simulink model "acf_rl_native"  (R2026b)
settings: Solver=ode4  StopTime=inf  FixedStep=3.3333333333333333e-06
InitFcn:
  | acf_select_actuator(bdroot);
model workspace (MAT data in the model file):
  acfControlVersion = 'force-observer-v1'
  acfImplementation = 'simple'
  acfLayoutVersion = 1
  p : object (value not decoded)
  pCompliant.actuator.kind = 'voice_coil'
  pCompliant.sim.step = 5e-05
  pCompliant.sim.stopTime = 4
  pCompliant.sim.evaluateFrom = 0
  pCompliant.force.reference = 20
  pCompliant.force.tolerance = 0.5
  pCompliant.force.sampleTime = 0.0001
  pCompliant.force.antiWindupRate = 30
  pCompliant.force.derivativeFilter = 0.001
  pCompliant.mechanics.mA = 0.4
  pCompliant.mechanics.mB = 0.6
  pCompliant.mechanics.mS = 1.4
  pCompliant.mechanics.k1 = 19746
  pCompliant.mechanics.k2 = 19746
  pCompliant.mechanics.c1 = 30
  pCompliant.mechanics.c2 = 5
  pCompliant.mechanics.gravity = 9.81
  pCompliant.mechanics.angle = 0
  pCompliant.mechanics.travelMin = 0
  pCompliant.mechanics.travelMax = 0.025
  pCompliant.mechanics.midTravel = 0.0125
  pCompliant.mechanics.lowerRigid = 0
  pCompliant.mechanics.upperRigid = 0
  pCompliant.robot.initialExcessForce = 10
  pCompliant.robot.sampleTime = 0.01
  pCompliant.robot.delay = 0.08
  pCompliant.robot.recenterGain = 0.8
  pCompliant.robot.deadband = 0.0005
  pCompliant.robot.responseTime = 0.06
  pCompliant.robot.maxSpeed = 0.02
  pCompliant.robot.maxAcceleration = 0.5
  pCompliant.robot.nominalVelocity = 0.005
  pCompliant.robot.errorRiseTime = 0.2
  pCompliant.robot.errorForce = 20
  pCompliant.robot.forceGate.enabled = 1
  pCompliant.robot.forceGate.errorBand_N = 0.2
  pCompliant.robot.forceGate.maxRate_N_s = 2
  pCompliant.robot.forceGate.dwellTime = 0.1
  pCompliant.robot.forceGate.filterTime = 0.1
  pCompliant.robot.forceGate.maxDelayGainProduct = 0.25
  pCompliant.robot.initialPositionOffset_m = 0
  pCompliant.sensor.sampleTime = 0.0001
  pCompliant.sensor.filterTime = 0.0001
  pCompliant.sensor.delay = 0.0001
  pCompliant.sensor.bias = 0
  pCompliant.sensor.noiseRms = 0.02
  pCompliant.sensor.seed = 1729
  pCompliant.sensor.strokeNoiseRms = 1e-06
  pCompliant.sensor.strokeDelay = 0.0001
  pCompliant.sensor.distalMass_kg = 1.4
  pCompliant.sensor.distalMass_model_kg = 1.4
  pCompliant.sensor.strokeBias = 0
  pCompliant.sensor.positionTarget = 'tool_relative_A'
  pCompliant.sensor.positionModel = 1
  pCompliant.surface.kind = 'sharp_bump'
  pCompliant.surface.startTime = 2
  pCompliant.surface.height = 0.001
  pCompliant.surface.width = 0.01
  pCompliant.surface.scanSpeed = 0.1
  pCompliant.surface.repeatPeriod = 1.2
  pCompliant.screw.lead = 0.01
  pCompliant.screw.rotorInertia = 5e-06
  pCompliant.screw.torqueConstant = 0.05
  pCompliant.screw.backEmfConstant = 0.05
  pCompliant.screw.resistance = 1
  pCompliant.screw.inductance = 0.001
  pCompliant.screw.peakCurrent = 5
  pCompliant.screw.voltage = 36
  pCompliant.screw.currentResponse = 0.001
  pCompliant.screw.coulombTorque = 0.004
  pCompliant.screw.viscousTorque = 2e-05
  pCompliant.screw.frictionSpeed = 0.2
  pCompliant.screw.speedBandwidth = 600
  pCompliant.screw.speedDamping = 1
  pCompliant.screw.speedAntiWindup = 100
  pCompliant.screw.maxLinearSpeedRequest = 0.1
  pCompliant.screw.forceKp = 0.08
  pCompliant.screw.forceKi = 0.5
  pCompliant.screw.forceKd = 0
  pCompliant.coil.forceConstant = 20
  pCompliant.coil.resistance = 4
  pCompliant.coil.inductance = 0.003
  pCompliant.coil.peakCurrent = 3.5
  pCompliant.coil.voltage = 24
  pCompliant.coil.currentResponse = 0.0001
  pCompliant.coil.coulombForce = 0.2
  pCompliant.coil.viscousFriction = 2
  pCompliant.coil.frictionSpeed = 0.0002
  pCompliant.coil.control.forceScale_N = 0.08
  pCompliant.coil.control.integralScale_Ns = 0.02
  pCompliant.coil.control.velocityScale_m_s = 0.1
  pCompliant.coil.control.currentScale_A = 1
  pCompliant.coil.control.surfaceJerkPower = 30
  pCompliant.coil.control.robotJerkPower = 0.2
  pCompliant.coil.control.forceNoise_N = 0.06
  pCompliant.coil.control.strokeNoise_m = 1e-06
  pCompliant.coil.control.frictionPower = 0.0009
  pCompliant.coil.strategy = 'observer'
  pCompliant.coil.forceKp = 0.03
  pCompliant.coil.forceKi = 20
  pCompliant.coil.forceKd = 5e-06
  pCompliant.coil.derivativeFilter = 0.0003
  pCompliant.coil.directCoulombCorrection = 1
  pCompliant.ideal.positionGain = 100
  pCompliant.ideal.velocityTime = 0.005
  pCompliant.ideal.maxSpeed = 0.1
  pCompliant.ideal.maxAcceleration = 20
  pCompliant.ideal.maxAxialForce = Inf
  pCompliant.ideal.forceKp = 7.49999999996e-05
  pCompliant.ideal.forceKi = 0.0179999999999
  pCompliant.ideal.forceKd = 0
  pCompliant.d.M = 1
  pCompliant.d.alpha = 0.4
  pCompliant.d.beta = 0.6
  pCompliant.d.mu = 0.24
  pCompliant.d.g = 9.81
  pCompliant.d.keq = 9873
  pCompliant.d.ell = 0.00159154943092
  pCompliant.d.q10 = 6.266
  pCompliant.d.q20 = -3.544
  pCompliant.d.holdForce = 0.38
  pCompliant.d.r0 = -0.00101286336473
  pCompliant.d.u0 = -0.00101286336473
  pCompliant.d.z0 = -0.000405145345893
  pCompliant.d.forceTicks = 2
  pCompliant.d.sensorTicks = 2
  pCompliant.d.robotTicks = 200
  pCompliant.d.sensorDelaySamples = 1
  pCompliant.d.robotDelaySamples = 8
  pCompliant.d.strokeDelaySamples = 1
  pCompliant.d.duration = 0.1
  pCompliant.d.screwHoldCurrent = 0.012095775675
  pCompliant.d.coilHoldCurrent = 0.019
  pCompliant.d.speedKp = 0.134590250444
  pCompliant.d.speedKi = 40.3770751333
  pCompliant.d.forceKp = 0.03
  pCompliant.d.forceKi = 20
  pCompliant.d.forceFeedforward = 0.019
  pCompliant.d.commandMax = 3.5
  pCompliant.d.commandMin = -3.5
  pCompliant.d.coilControl.A = [0.999835746645  0.00997449730862  2.7375365216e-08  7.61651197841e-10  0  -1.6633847877e-06  0.000122366168772  4.99154092539e-05  -1.86997975018e-12  -0.00413675380364  0.0458269373325; -0.0328205964433  0.994849329683  8.20753911342e-06  2.35203256889e-07  0  -0.000332344666304  0.0209978497532  0.00997449730862  -7.61339530061e-10  -0.0648188925165  1.4845666459; 2.73753650079e-08  4.2275891689e-09  0.999753329061  0.00999293153119  0  -2.49816229398e-06  0.000183793671919  1.05385993767e-11  -4.99493633224e-05  -0.00412753174604  0.239523975118; 8.20753911342e-06  1.27434271721e-06  -0.0493177743256  0.99850452489  0  -0.000499438537288  0.0315644865369  4.22758920489e-09  -0.00998460663731  -0.0815985605483  3.59792231768; -0.00016422598009  -2.54984637932e-05  -0.000246643563285  -7.06770715559e-06  1  0.00999583845292  0.000306159840692  -8.45802075454e-08  2.28686000246e-08  -0.00684940440528  0.403167864802; -0.0328123889042  -0.00514939597465  -0.0493095667865  -0.00149523990651  0  0.999168216796  0.05256233629  -2.54984637932e-05  7.06389572225e-06  -0.13409460151  6.02904033295; 0  0  0  0  0  0  0.367879441171  0  0  -7.97431898094e-16  1.21101563191e-14; 0  0  0  0  0  0  0  1  0  -0.0527908571517  -3.83687930661; 0  0  0  0  0  0  0  0  0.998334721451  -1.1298863089e-06  6.97113672767e-05; 12.4818525546  1.89636167649  0  0  0  0  0  0  0  0.118421048821  5.02664399852; 1  0  0  0  -1  0  0  0  0  0.00201545569863  -0.311994254342]
  pCompliant.d.coilControl.B = [0.00413675380364  -45.8269373325  4.39723099978e-05  -8.31692393848e-06  -1.87066620522e-13; 0.0648188925165  -1484.5666459  0.0122366168773  -0.00166172333152  -7.61651187423e-11; 0.00412753174604  -239.523975118  6.60225574786e-05  -1.24908114699e-05  -4.99771201703e-06; 0.0815985605483  -3597.92231768  0.018379367192  -0.00249719268644  -0.000999293153119; 0.00684940440528  -403.167864802  0.000109994867477  -2.08077354085e-05  2.28779591191e-09; 0.13409460151  -6029.04033295  0.0306159840692  -0.00415891601796  7.06770715559e-07; 7.97431898094e-16  -1.21101563191e-11  0.632120558829  0  0; 0.0527908571517  3836.87930661  0  0  0; 1.1298863089e-06  -0.0697113672767  0  0  0; 0.24945839235  -5026.64399852  0  0  0; -0.00201545569863  311.994254342  0  0  0]
  pCompliant.d.coilControl.C = [0.001  0  0  0  0  0  0  0  0  -3.48871506098e-06  3.07351175913e-05; 0  0.1  0  0  0  0  0  0  0  -0.00647853206073  0.153375714294; 0  0  0.001  0  0  0  0  0  0  -3.3097478138e-06  0.000203450968232; 0  0  0  0.1  0  0  0  0  0  -0.00819516417082  0.361638855458; 0  0  0  0  0.001  0  0  0  0  -5.5041707596e-06  0.000342729371933; 0  0  0  0  0  0.1  0  0  0  -0.0134942008024  0.605832757613; 0  0  0  0  0  0  1  0  0  -2.16764463802e-15  3.2918817862e-14; 0  0  0  0  0  0  0  10  0  -0.527908571517  -38.3687930661; 0  0  0  0  0  0  0  0  10  -1.13177102291e-05  0.00069827649764]
  pCompliant.d.coilControl.D = [3.48871506098e-06  -0.0307351175913  0  0  0; 0.00647853206073  -153.375714294  0  0  0; 3.3097478138e-06  -0.203450968232  0  0  0; 0.00819516417082  -361.638855458  0  0  0; 5.5041707596e-06  -0.342729371933  0  0  0; 0.0134942008024  -605.832757613  0  0  0; 2.16764463802e-15  -3.2918817862e-11  0  0  0; 0.527908571517  38368.7930661  0  0  0; 1.13177102291e-05  -0.69827649764  0  0  0]
  pCompliant.d.coilControl.feedback = [-244976.099879 -409.158583232 -93.7245887968 0.421195616079 0 0 -0.929640363397 -17.5713692327 -0.00189860404734]
  pCompliant.d.coilControl.integralGain = 50
  pCompliant.d.coilControl.force = [19746 30 0 0 0 0 0 1.4 0]
  pCompliant.d.recenterGain = 0.735294117647
  pCompliant.d.positionMeasurementBias = -0.0135128633647
  pCompliant.d.positionMeasurementInitial = 0.0135128633647
  pCompliant.d.forceKd = 0
  pCompliant.d.derivativeFilter = 0.0003
  pCompliant.springs.maxCombinedLength_m = 0.1
  pCompliant.springs.commonPreload_N = 34
  pCompliant.springs.workingClearance_m = 0.0005
  pCompliant.springs.unseatingClearance_m = 0.00025
  pCompliant.springs.lower.part = 'D-180S'
  pCompliant.springs.lower.rate_N_m = 9873
  pCompliant.springs.lower.freeLength_m = 0.0181
  pCompliant.springs.lower.freeLengthTolerance_m = 0.00049
  pCompliant.springs.lower.minWorkingLength_m = 0.01055
  pCompliant.springs.lower.maxCyclicStroke_m = 0.00318
  pCompliant.springs.lower.forceEnvelope_N = 68.543
  pCompliant.springs.upper.part = 'D-180S'
  pCompliant.springs.upper.rate_N_m = 9873
  pCompliant.springs.upper.freeLength_m = 0.0181
  pCompliant.springs.upper.freeLengthTolerance_m = 0.00049
  pCompliant.springs.upper.minWorkingLength_m = 0.01055
  pCompliant.springs.upper.maxCyclicStroke_m = 0.00318
  pCompliant.springs.upper.forceEnvelope_N = 68.543
  pCompliant.robotPrediction.enabled = 1
  pCompliant.robotPrediction.delay = 0.08
  pCompliant.robotPrediction.responseTime = 0.06
  pCompliant.robotPrediction.maxSpeed = 0.02
  pCompliant.robotPrediction.maxAcceleration = 0.5
  pCompliant.robotPrediction.residualTime = 0.06
  pCompliant.robotPrediction.residualJerkPower = 0.0002
  pCompliant.robotPrediction.boundedNominalPath = 1
  pCompliant.robotPrediction.delaySamples = 8
  pCompliant.robotPrediction.surfaceJerkEnabled = 0
  pCompliant.robotPrediction.surfaceSnapPower = 1000000
  pCompliant.robotPrediction.surfaceJerkDecayTime = Inf
  pCompliant.robotPrediction.surfaceJerkFeedforwardGain = 0
  pNearContact.actuator.kind = 'voice_coil'
  pNearContact.sim.step = 0.0001
  pNearContact.sim.stopTime = 4
  pNearContact.sim.evaluateFrom = 0
  pNearContact.force.reference = 20
  pNearContact.force.tolerance = 0.5
  pNearContact.force.sampleTime = 0.0002
  pNearContact.force.antiWindupRate = 30
  pNearContact.force.derivativeFilter = 0.001
  pNearContact.mechanics.mA = 0.4
  pNearContact.mechanics.mB = 0.6
  pNearContact.mechanics.mS = 1.4
  pNearContact.mechanics.k1 = 19746
  pNearContact.mechanics.k2 = 0
  pNearContact.mechanics.c1 = 60
  pNearContact.mechanics.c2 = 0
  pNearContact.mechanics.gravity = 9.81
  pNearContact.mechanics.angle = 0
  pNearContact.mechanics.travelMin = 0
  pNearContact.mechanics.travelMax = 0.025
  pNearContact.mechanics.midTravel = 0.0125
  pNearContact.mechanics.lowerRigid = 0
  pNearContact.mechanics.upperRigid = 1
  pNearContact.robot.initialExcessForce = 10
  pNearContact.robot.sampleTime = 0.01
  pNearContact.robot.delay = 0.08
  pNearContact.robot.recenterGain = 0.8
  pNearContact.robot.deadband = 0.0005
  pNearContact.robot.responseTime = 0.06
  pNearContact.robot.maxSpeed = 0.02
  pNearContact.robot.maxAcceleration = 0.5
  pNearContact.robot.nominalVelocity = 0
  pNearContact.robot.errorRiseTime = 0.2
  pNearContact.robot.errorForce = 20
  pNearContact.robot.forceGate.enabled = 1
  pNearContact.robot.forceGate.errorBand_N = 0.2
  pNearContact.robot.forceGate.maxRate_N_s = 2
  pNearContact.robot.forceGate.dwellTime = 0.1
  pNearContact.robot.forceGate.filterTime = 0.02
  pNearContact.robot.forceGate.maxDelayGainProduct = 0.25
  pNearContact.robot.initialPositionOffset_m = 0
  pNearContact.sensor.sampleTime = 0.0002
  pNearContact.sensor.filterTime = 0.0003
  pNearContact.sensor.delay = 0
  pNearContact.sensor.bias = 0
  pNearContact.sensor.noiseRms = 0
  pNearContact.sensor.seed = 1729
  pNearContact.sensor.strokeNoiseRms = 1e-06
  pNearContact.sensor.strokeDelay = 0.0002
  pNearContact.sensor.distalMass_kg = 0
  pNearContact.sensor.distalMass_model_kg = 0
  pNearContact.sensor.positionModel = 0
  pNearContact.sensor.positionTarget = 'magnet_gap'
  pNearContact.surface.kind = 'sharp_bump'
  pNearContact.surface.startTime = 2
  pNearContact.surface.height = 0.001
  pNearContact.surface.width = 0.01
  pNearContact.surface.scanSpeed = 0.1
  pNearContact.surface.repeatPeriod = 1.2
  pNearContact.screw.lead = 0.005
  pNearContact.screw.rotorInertia = 2e-05
  pNearContact.screw.torqueConstant = 0.05
  pNearContact.screw.backEmfConstant = 0.05
  pNearContact.screw.resistance = 1
  pNearContact.screw.inductance = 0.001
  pNearContact.screw.peakCurrent = 3
  pNearContact.screw.voltage = 24
  pNearContact.screw.currentResponse = 0.001
  pNearContact.screw.coulombTorque = 0.004
  pNearContact.screw.viscousTorque = 2e-05
  pNearContact.screw.frictionSpeed = 0.2
  pNearContact.screw.speedBandwidth = 150
  pNearContact.screw.speedDamping = 1
  pNearContact.screw.speedAntiWindup = 100
  pNearContact.screw.maxLinearSpeedRequest = 0.1
  pNearContact.screw.forceKp = 0.02
  pNearContact.screw.forceKi = 0.008
  pNearContact.screw.forceKd = 0
  pNearContact.coil.forceConstant = 20
  pNearContact.coil.resistance = 4
  pNearContact.coil.inductance = 0.003
  pNearContact.coil.peakCurrent = 3
  pNearContact.coil.voltage = 24
  pNearContact.coil.currentResponse = 0.0004
  pNearContact.coil.coulombForce = 0.2
  pNearContact.coil.viscousFriction = 2
  pNearContact.coil.frictionSpeed = 0.0002
  pNearContact.coil.control.forceScale_N = 0.04
  pNearContact.coil.control.integralScale_Ns = 0.02
  pNearContact.coil.control.velocityScale_m_s = 0.1
  pNearContact.coil.control.currentScale_A = 1
  pNearContact.coil.control.surfaceJerkPower = 70
  pNearContact.coil.control.robotJerkPower = 0.2
  pNearContact.coil.control.forceNoise_N = 0.06
  pNearContact.coil.control.strokeNoise_m = 1e-06
  pNearContact.coil.control.frictionPower = 0.0009
  pNearContact.coil.strategy = 'observer'
  pNearContact.coil.forceKp = 0.64
  pNearContact.coil.forceKi = 300
  pNearContact.coil.forceKd = 0.0006
  pNearContact.coil.derivativeFilter = 0.0002
  pNearContact.coil.directCoulombCorrection = 0
  pNearContact.ideal.positionGain = 100
  pNearContact.ideal.velocityTime = 0.005
  pNearContact.ideal.maxSpeed = 0.1
  pNearContact.ideal.maxAcceleration = 20
  pNearContact.ideal.maxAxialForce = Inf
  pNearContact.ideal.forceKp = 7.49999999996e-05
  pNearContact.ideal.forceKi = 0.0179999999999
  pNearContact.ideal.forceKd = 0
  pNearContact.d.M = 1
  pNearContact.d.alpha = 0.4
  pNearContact.d.beta = 0.6
  pNearContact.d.mu = 0.24
  pNearContact.d.g = 9.81
  pNearContact.d.keq = 19746
  pNearContact.d.ell = 0.000795774715459
  pNearContact.d.q10 = 6.266
  pNearContact.d.q20 = -3.544
  pNearContact.d.holdForce = 0.38
  pNearContact.d.r0 = -0.000506431682366
  pNearContact.d.u0 = -0.000506431682366
  pNearContact.d.z0 = -0.000202572672946
  pNearContact.d.forceTicks = 2
  pNearContact.d.sensorTicks = 2
  pNearContact.d.robotTicks = 100
  pNearContact.d.sensorDelaySamples = 0
  pNearContact.d.robotDelaySamples = 8
  pNearContact.d.strokeDelaySamples = 1
  pNearContact.d.duration = 0.1
  pNearContact.d.screwHoldCurrent = 0.00604788783749
  pNearContact.d.coilHoldCurrent = 0.019
  pNearContact.d.speedKp = 0.120911890653
  pNearContact.d.speedKi = 9.06839179896
  pNearContact.d.forceKp = 0.64
  pNearContact.d.forceKi = 300
  pNearContact.d.forceFeedforward = 0.019
  pNearContact.d.commandMax = 3
  pNearContact.d.commandMin = -3
  pNearContact.d.coilControl.A = [1.0026534079  0.0208018967614  0  0  0  -6.62025176034e-06  0.000564047674022  0.00254334714763  -4.42128553796e-08  0.000176714388546  -0.204677748701; -0.237328903655  0.927231856972  0  0  0  -0.00065968023534  0.0518668316835  -0.102292582547  -6.62025176034e-06  -0.00920161779651  -4.36343291704; 0  0  0.818730753078  0  0  0  0  0  0  0  0; 0  0  0  0.818730753078  0  0  0  0  0  0  0; -0.00626191608391  -0.00190710475355  0  0  1  0.0199933797482  0.000564047674022  -0.0039776563872  0.000199955787144  -0.000299685353291  -0.591080531092; -0.205759420553  -0.0631754711644  0  0  0  0.999340319765  0.0518668316835  -0.0999096815332  0.0199933797482  -0.0075146691647  -4.76194052863; -7.21925622066e-14  -2.19363604396e-14  0  0  0  0  0.606530659713  -5.11848410256e-14  0  -3.85768571654e-15  -5.1788789238e-13; -0.870024269621  -0.264364712738  0  0  0  0  0  0.383149003611  0  -0.046490664625  2.07853967939; -0.0101705012363  -0.00309039843096  0  0  0  0  0  -0.00721092967225  1  -0.000543471462297  -0.478477076797; 2.12271455447  0.645005941801  0  0  0  0  0  1.5050138642  0  0.113429491443  -0.281433751395; -0.00276622884074  -0.000840543555375  0  0  1  0  0  -0.00196126829588  0  -0.000147816356165  -0.494907709778]
  pNearContact.d.coilControl.B = [-0.000344192630114  204.677748701  9.79775020114e-05  -3.31012588017e-05  0; 0.017922304215  4363.43291704  0.0141011918506  -0.0032984011767  0; 0  0  0  0  0; 0  0  0  0  0; 0.00058370736421  591.080531092  9.79775020113e-05  -3.31012588017e-05  0; 0.0146365769394  4761.94052863  0.0141011918506  -0.0032984011767  0; 7.5137457898e-15  5.1788789238e-10  0.393469340287  0  0; 0.0905514500813  -2078.53967939  0  0  0; 0.00105853786746  478.477076797  0  0  0; 0.779069518257  281.433751395  0  0  0; 0.000287906948728  494.907709778  0  0  0]
  pNearContact.d.coilControl.C = [0.00100660851405  2.00805653396e-06  0  0  0  0  0  4.6854652459e-06  0  3.53132919675e-07  -0.000115963676268; -0.0157866520328  0.0952030835513  0  0  0  0  0  -0.011192805047  0  -0.000843576404514  -0.450749165677; 0  0  0.001  0  0  0  0  0  0  0  0; 0  0  0  0.1  0  0  0  0  0  0  0; -2.76622884074e-06  -8.40543555375e-07  0  0  0.001  0  0  -1.96126829588e-06  0  -1.47816356165e-07  -0.000494907709778; -0.0143494112594  -0.00436019789102  0  0  0  0.1  0  -0.0101737950791  0  -0.000766775927659  -0.485485893323; -1.19025412896e-13  -3.61669440584e-14  0  0  0  0  1  -8.43895361364e-14  0  -6.36024849654e-15  -8.53852784006e-13; -8.70024269621  -2.64364712738  0  0  0  0  0  3.83149003611  0  -0.46490664625  20.7853967939; -0.101705012363  -0.0309039843096  0  0  0  0  0  -0.0721092967225  10  -0.00543471462297  -4.78477076797]
  pNearContact.d.coilControl.D = [-6.87809008668e-07  0.115963676268  0  0  0; 0.0016430624793  450.749165677  0  0  0; 0  0  0  0  0; 0  0  0  0  0; 2.87906948728e-07  0.494907709778  0  0  0; 0.00149347557616  485.485893323  0  0  0; 1.23880725063e-14  8.53852784006e-10  0  0  0; 0.905514500813  -20785.3967939  0  0  0; 0.0105853786746  4784.77076797  0  0  0]
  pNearContact.d.coilControl.feedback = [-138262.14092 -455.642921278 0 0 0 0 -2.78835552108 -10.1816815608 0]
  pNearContact.d.coilControl.integralGain = 14.3726319371
  pNearContact.d.coilControl.force = [19746 60 0 0 0 0 0 1.4 0]
  pNearContact.d.recenterGain = 0.8
  pNearContact.d.forceKd = 0
  pNearContact.d.derivativeFilter = 0.0002
  pNearContact.d.positionMeasurementBias = -0.0119935683176
  pNearContact.d.positionMeasurementInitial = 0.0119935683176
  pNearContact.springs.maxCombinedLength_m = 0.1
  pNearContact.springs.commonPreload_N = 32
  pNearContact.springs.workingClearance_m = 0.0005
  pNearContact.springs.unseatingClearance_m = 0.00025
  pNearContact.springs.lower.part = 'D-180S'
  pNearContact.springs.lower.rate_N_m = 9873
  pNearContact.springs.lower.freeLength_m = 0.0181
  pNearContact.springs.lower.freeLengthTolerance_m = 0.00049
  pNearContact.springs.lower.minWorkingLength_m = 0.01055
  pNearContact.springs.lower.maxCyclicStroke_m = 0.00318
  pNearContact.springs.lower.forceEnvelope_N = 68.543
  pNearContact.springs.upper.part = 'D-180N'
  pNearContact.springs.upper.rate_N_m = 3673
  pNearContact.springs.upper.freeLength_m = 0.0228
  pNearContact.springs.upper.freeLengthTolerance_m = 0.00075
  pNearContact.springs.upper.minWorkingLength_m = 0.00815
  pNearContact.springs.upper.maxCyclicStroke_m = 0.00536
  pNearContact.springs.upper.forceEnvelope_N = 50.267
  pNearContact.robotPrediction.enabled = 0
  pNearContact.robotPrediction.delay = 0.08
  pNearContact.robotPrediction.responseTime = 0.06
  pNearContact.robotPrediction.maxSpeed = 0.02
  pNearContact.robotPrediction.maxAcceleration = 0.5
  pNearContact.robotPrediction.residualTime = 0.06
  pNearContact.robotPrediction.residualJerkPower = 0.0002
  pNearContact.robotPrediction.boundedNominalPath = 0
  pNearContact.robotPrediction.delaySamples = 8
  pNoSprings.actuator.kind = 'voice_coil'
  pNoSprings.sim.step = 5e-05
  pNoSprings.sim.stopTime = 4
  pNoSprings.sim.evaluateFrom = 0
  pNoSprings.force.reference = 20
  pNoSprings.force.tolerance = 0.5
  pNoSprings.force.sampleTime = 0.0001
  pNoSprings.force.antiWindupRate = 30
  pNoSprings.force.derivativeFilter = 0.001
  pNoSprings.mechanics.mA = 0.4
  pNoSprings.mechanics.mB = 0.6
  pNoSprings.mechanics.mS = 1.4
  pNoSprings.mechanics.k1 = 0
  pNoSprings.mechanics.k2 = 0
  pNoSprings.mechanics.c1 = 0
  pNoSprings.mechanics.c2 = 0
  pNoSprings.mechanics.gravity = 9.81
  pNoSprings.mechanics.angle = 0
  pNoSprings.mechanics.travelMin = 0
  pNoSprings.mechanics.travelMax = 0.025
  pNoSprings.mechanics.midTravel = 0.0125
  pNoSprings.mechanics.lowerRigid = 1
  pNoSprings.mechanics.upperRigid = 1
  pNoSprings.robot.initialExcessForce = 10
  pNoSprings.robot.sampleTime = 0.01
  pNoSprings.robot.delay = 0.08
  pNoSprings.robot.recenterGain = 0.8
  pNoSprings.robot.deadband = 0.0005
  pNoSprings.robot.responseTime = 0.06
  pNoSprings.robot.maxSpeed = 0.02
  pNoSprings.robot.maxAcceleration = 0.5
  pNoSprings.robot.nominalVelocity = 0.005
  pNoSprings.robot.errorRiseTime = 0.2
  pNoSprings.robot.errorForce = 20
  pNoSprings.robot.forceGate.enabled = 1
  pNoSprings.robot.forceGate.errorBand_N = 0.2
  pNoSprings.robot.forceGate.maxRate_N_s = 2
  pNoSprings.robot.forceGate.dwellTime = 0.1
  pNoSprings.robot.forceGate.filterTime = 0.1
  pNoSprings.robot.forceGate.maxDelayGainProduct = 0.25
  pNoSprings.robot.initialPositionOffset_m = 0
  pNoSprings.sensor.sampleTime = 0.0001
  pNoSprings.sensor.filterTime = 0.0001
  pNoSprings.sensor.delay = 0.0001
  pNoSprings.sensor.bias = 0
  pNoSprings.sensor.noiseRms = 0.02
  pNoSprings.sensor.seed = 1729
  pNoSprings.sensor.strokeNoiseRms = 1e-06
  pNoSprings.sensor.strokeDelay = 0.0001
  pNoSprings.sensor.distalMass_kg = 1.4
  pNoSprings.sensor.distalMass_model_kg = 1.4
  pNoSprings.sensor.strokeBias = 0
  pNoSprings.sensor.positionTarget = 'tool_relative_A'
  pNoSprings.sensor.positionModel = 1
  pNoSprings.surface.kind = 'sharp_bump'
  pNoSprings.surface.startTime = 2
  pNoSprings.surface.height = 0.001
  pNoSprings.surface.width = 0.01
  pNoSprings.surface.scanSpeed = 0.1
  pNoSprings.surface.repeatPeriod = 1.2
  pNoSprings.screw.lead = 0.01
  pNoSprings.screw.rotorInertia = 5e-06
  pNoSprings.screw.torqueConstant = 0.05
  pNoSprings.screw.backEmfConstant = 0.05
  pNoSprings.screw.resistance = 1
  pNoSprings.screw.inductance = 0.001
  pNoSprings.screw.peakCurrent = 5
  pNoSprings.screw.voltage = 36
  pNoSprings.screw.currentResponse = 0.001
  pNoSprings.screw.coulombTorque = 0.004
  pNoSprings.screw.viscousTorque = 2e-05
  pNoSprings.screw.frictionSpeed = 0.2
  pNoSprings.screw.speedBandwidth = 600
  pNoSprings.screw.speedDamping = 1
  pNoSprings.screw.speedAntiWindup = 100
  pNoSprings.screw.maxLinearSpeedRequest = 0.1
  pNoSprings.screw.forceKp = 0.08
  pNoSprings.screw.forceKi = 0.5
  pNoSprings.screw.forceKd = 0
  pNoSprings.coil.forceConstant = 20
  pNoSprings.coil.resistance = 4
  pNoSprings.coil.inductance = 0.003
  pNoSprings.coil.peakCurrent = 3.5
  pNoSprings.coil.voltage = 24
  pNoSprings.coil.currentResponse = 0.0001
  pNoSprings.coil.coulombForce = 0.2
  pNoSprings.coil.viscousFriction = 2
  pNoSprings.coil.frictionSpeed = 0.0002
  pNoSprings.coil.control.forceScale_N = 0.32
  pNoSprings.coil.control.integralScale_Ns = 0.02
  pNoSprings.coil.control.velocityScale_m_s = 0.1
  pNoSprings.coil.control.currentScale_A = 1
  pNoSprings.coil.control.surfaceJerkPower = 70
  pNoSprings.coil.control.robotJerkPower = 0.2
  pNoSprings.coil.control.forceNoise_N = 0.02
  pNoSprings.coil.control.strokeNoise_m = 1e-06
  pNoSprings.coil.control.frictionPower = 0.0009
  pNoSprings.coil.strategy = 'observer'
  pNoSprings.coil.forceKp = 0.03
  pNoSprings.coil.forceKi = 20
  pNoSprings.coil.forceKd = 5e-06
  pNoSprings.coil.derivativeFilter = 0.0003
  pNoSprings.coil.directCoulombCorrection = 1
  pNoSprings.ideal.positionGain = 100
  pNoSprings.ideal.velocityTime = 0.005
  pNoSprings.ideal.maxSpeed = 0.1
  pNoSprings.ideal.maxAcceleration = 20
  pNoSprings.ideal.maxAxialForce = Inf
  pNoSprings.ideal.forceKp = 7.49999999996e-05
  pNoSprings.ideal.forceKi = 0.0179999999999
  pNoSprings.ideal.forceKd = 0
  pNoSprings.d.M = 1
  pNoSprings.d.alpha = 0.4
  pNoSprings.d.beta = 0.6
  pNoSprings.d.mu = 0.24
  pNoSprings.d.g = 9.81
  pNoSprings.d.keq = Inf
  pNoSprings.d.ell = 0.00159154943092
  pNoSprings.d.q10 = 6.266
  pNoSprings.d.q20 = -3.544
  pNoSprings.d.holdForce = 0.38
  pNoSprings.d.r0 = 0
  pNoSprings.d.u0 = 0
  pNoSprings.d.z0 = 0
  pNoSprings.d.forceTicks = 2
  pNoSprings.d.sensorTicks = 2
  pNoSprings.d.robotTicks = 200
  pNoSprings.d.sensorDelaySamples = 1
  pNoSprings.d.robotDelaySamples = 8
  pNoSprings.d.strokeDelaySamples = 1
  pNoSprings.d.duration = 0.1
  pNoSprings.d.screwHoldCurrent = 0.012095775675
  pNoSprings.d.coilHoldCurrent = 0.019
  pNoSprings.d.speedKp = 0.134590250444
  pNoSprings.d.speedKi = 40.3770751333
  pNoSprings.d.forceKp = 0.03
  pNoSprings.d.forceKi = 20
  pNoSprings.d.forceFeedforward = 0.019
  pNoSprings.d.commandMax = 3.5
  pNoSprings.d.commandMin = -3.5
  pNoSprings.d.coilControl.A = [0.904837418036  0  0  0  0  0  0  0  0  2.67588421391e-14  -3.29524891735e-09; 0  0.904837418036  0  0  0  0  0  0  0  0  0; 0  0  0.904837418036  0  0  0  0  0  0  0  0; 0  0  0  0.904837418036  0  0  0  0  0  0  0; 0  0  0  0  1  0.01  0  -5e-05  4.99722337924e-05  7.56047730874e-05  0.030764915469; 0  0  0  0  0  1  0  -0.01  0.00999167129437  0.00527845864875  0.0453783132776; 0  0  0  0  0  0  0.367879441171  0  0  -7.29404615433e-13  6.17194806769e-14; 0  0  0  0  0  0  0  1  0  -0.189432576756  0.00157759478786; 0  0  0  0  0  0  0  0  0.998334721451  -2.54541925038e-08  0.00774836045737; 0  0  0  0  0  -0.126424111766  12.6424111766  3.79272335297  0  -0.643457512844  -0.000911475458531; 1  0  0  0  -1  0  0  0  0  -3.22918141347e-05  -0.0303114447317]
  pNoSprings.d.coilControl.B = [-2.67588421391e-14  3.29524891735e-06  0  0  0; 0  0  0  0  0; 0  0  0  0  0; 0  0  0  0  0; -7.56047730874e-05  -30.764915469  0  0  5e-06; -0.00527845864875  -45.3783132776  0  0  0.001; 7.29404615433e-13  -6.17194806769e-11  0.632120558829  0  0; 0.189432576756  -1.57759478786  0  0  0; 2.54541925038e-08  -7.74836045737  0  0  0; 1.01133695401  0.911475458531  0  -0.632120558829  0; 3.22918141347e-05  30.3114447317  0  0  0]
  pNoSprings.d.coilControl.C = [0.001  0  0  0  0  0  0  0  0  2.95730941335e-17  -3.64181327127e-12; 0  0.1  0  0  0  0  0  0  0  0  0; 0  0  0.001  0  0  0  0  0  0  0  0; 0  0  0  0.1  0  0  0  0  0  0  0; 0  0  0  0  0.001  0  0  0  0  3.22918141643e-08  3.03114410899e-05; 0  0  0  0  0  0.1  0  0  0  0.000338413313594  0.00453165410154; 0  0  0  0  0  0  1  0  0  -1.98272731172e-12  1.67770942786e-13; 0  0  0  0  0  0  0  10  0  -1.89432576756  0.0157759478786; 0  0  0  0  0  0  0  0  10  -2.54966515307e-07  0.0776128515906]
  pNoSprings.d.coilControl.D = [-2.95730941335e-17  3.64181327127e-09  0  0  0; 0  0  0  0  0; 0  0  0  0  0; 0  0  0  0  0; -3.22918141643e-08  -0.0303114410899  0  0  0; -0.000338413313594  -4.53165410154  0  0  0; 1.98272731172e-12  -1.67770942786e-10  0  0  0; 1.89432576756  -15.7759478786  0  0  0; 2.54966515307e-07  -77.6128515906  0  0  0]
  pNoSprings.d.coilControl.feedback = [0 0 0 0 0 0 -0.584132933117 -0.158413293312 0]
  pNoSprings.d.coilControl.integralGain = 1.2641098067
  pNoSprings.d.coilControl.force = [0 0 0 0 0 -2 20 2 0]
  pNoSprings.d.recenterGain = 0.735294117647
  pNoSprings.d.positionMeasurementBias = -0.0125
  pNoSprings.d.positionMeasurementInitial = 0.0125
  pNoSprings.d.forceKd = 0
  pNoSprings.d.derivativeFilter = 0.0003
  pNoSprings.springs.maxCombinedLength_m = 0.1
  pNoSprings.springs.commonPreload_N = 32
  pNoSprings.springs.workingClearance_m = 0.0005
  pNoSprings.springs.unseatingClearance_m = 0.00025
  pNoSprings.springs.lower.part = 'D-180S'
  pNoSprings.springs.lower.rate_N_m = 9873
  pNoSprings.springs.lower.freeLength_m = 0.0181
  pNoSprings.springs.lower.freeLengthTolerance_m = 0.00049
  pNoSprings.springs.lower.minWorkingLength_m = 0.01055
  pNoSprings.springs.lower.maxCyclicStroke_m = 0.00318
  pNoSprings.springs.lower.forceEnvelope_N = 68.543
  pNoSprings.springs.upper.part = 'D-180S'
  pNoSprings.springs.upper.rate_N_m = 9873
  pNoSprings.springs.upper.freeLength_m = 0.0181
  pNoSprings.springs.upper.freeLengthTolerance_m = 0.00049
  pNoSprings.springs.upper.minWorkingLength_m = 0.01055
  pNoSprings.springs.upper.maxCyclicStroke_m = 0.00318
  pNoSprings.springs.upper.forceEnvelope_N = 68.543
  pNoSprings.robotPrediction.enabled = 1
  pNoSprings.robotPrediction.delay = 0.08
  pNoSprings.robotPrediction.responseTime = 0.06
  pNoSprings.robotPrediction.maxSpeed = 0.02
  pNoSprings.robotPrediction.maxAcceleration = 0.5
  pNoSprings.robotPrediction.residualTime = 0.06
  pNoSprings.robotPrediction.residualJerkPower = 0.0002
  pNoSprings.robotPrediction.boundedNominalPath = 1
  pNoSprings.robotPrediction.delaySamples = 8
  pNoSprings.robotPrediction.surfaceJerkEnabled = 0
  pNoSprings.robotPrediction.surfaceSnapPower = 1000000
  pNoSprings.robotPrediction.surfaceJerkDecayTime = Inf
  pNoSprings.robotPrediction.surfaceJerkFeedforwardGain = 0
  pRecommended.actuator.kind = 'voice_coil'
  pRecommended.sim.step = 5e-05
  pRecommended.sim.stopTime = 4
  pRecommended.sim.evaluateFrom = 0
  pRecommended.force.reference = 20
  pRecommended.force.tolerance = 0.5
  pRecommended.force.sampleTime = 0.0001
  pRecommended.force.antiWindupRate = 30
  pRecommended.force.derivativeFilter = 0.001
  pRecommended.mechanics.mA = 0.4
  pRecommended.mechanics.mB = 0.6
  pRecommended.mechanics.mS = 1.4
  pRecommended.mechanics.k1 = 0
  pRecommended.mechanics.k2 = 0
  pRecommended.mechanics.c1 = 0
  pRecommended.mechanics.c2 = 0
  pRecommended.mechanics.gravity = 9.81
  pRecommended.mechanics.angle = 0
  pRecommended.mechanics.travelMin = 0
  pRecommended.mechanics.travelMax = 0.025
  pRecommended.mechanics.midTravel = 0.0125
  pRecommended.mechanics.lowerRigid = 1
  pRecommended.mechanics.upperRigid = 1
  pRecommended.robot.initialExcessForce = 10
  pRecommended.robot.sampleTime = 0.01
  pRecommended.robot.delay = 0.08
  pRecommended.robot.recenterGain = 0.8
  pRecommended.robot.deadband = 0.0005
  pRecommended.robot.responseTime = 0.06
  pRecommended.robot.maxSpeed = 0.02
  pRecommended.robot.maxAcceleration = 0.5
  pRecommended.robot.nominalVelocity = 0.005
  pRecommended.robot.errorRiseTime = 0.2
  pRecommended.robot.errorForce = 20
  pRecommended.robot.forceGate.enabled = 1
  pRecommended.robot.forceGate.errorBand_N = 0.2
  pRecommended.robot.forceGate.maxRate_N_s = 2
  pRecommended.robot.forceGate.dwellTime = 0.1
  pRecommended.robot.forceGate.filterTime = 0.1
  pRecommended.robot.forceGate.maxDelayGainProduct = 0.25
  pRecommended.robot.initialPositionOffset_m = 0
  pRecommended.sensor.sampleTime = 0.0001
  pRecommended.sensor.filterTime = 0.0001
  pRecommended.sensor.delay = 0.0001
  pRecommended.sensor.bias = 0
  pRecommended.sensor.noiseRms = 0.02
  pRecommended.sensor.seed = 1729
  pRecommended.sensor.strokeNoiseRms = 1e-06
  pRecommended.sensor.strokeDelay = 0.0001
  pRecommended.sensor.distalMass_kg = 1.4
  pRecommended.sensor.distalMass_model_kg = 1.4
  pRecommended.sensor.strokeBias = 0
  pRecommended.sensor.positionTarget = 'tool_relative_A'
  pRecommended.sensor.positionModel = 1
  pRecommended.surface.kind = 'sharp_bump'
  pRecommended.surface.startTime = 2
  pRecommended.surface.height = 0.001
  pRecommended.surface.width = 0.01
  pRecommended.surface.scanSpeed = 0.1
  pRecommended.surface.repeatPeriod = 1.2
  pRecommended.screw.lead = 0.01
  pRecommended.screw.rotorInertia = 5e-06
  pRecommended.screw.torqueConstant = 0.05
  pRecommended.screw.backEmfConstant = 0.05
  pRecommended.screw.resistance = 1
  pRecommended.screw.inductance = 0.001
  pRecommended.screw.peakCurrent = 5
  pRecommended.screw.voltage = 36
  pRecommended.screw.currentResponse = 0.001
  pRecommended.screw.coulombTorque = 0.004
  pRecommended.screw.viscousTorque = 2e-05
  pRecommended.screw.frictionSpeed = 0.2
  pRecommended.screw.speedBandwidth = 600
  pRecommended.screw.speedDamping = 1
  pRecommended.screw.speedAntiWindup = 100
  pRecommended.screw.maxLinearSpeedRequest = 0.1
  pRecommended.screw.forceKp = 0.08
  pRecommended.screw.forceKi = 0.5
  pRecommended.screw.forceKd = 0
  pRecommended.coil.forceConstant = 20
  pRecommended.coil.resistance = 4
  pRecommended.coil.inductance = 0.003
  pRecommended.coil.peakCurrent = 3.5
  pRecommended.coil.voltage = 24
  pRecommended.coil.currentResponse = 0.0001
  pRecommended.coil.coulombForce = 0.2
  pRecommended.coil.viscousFriction = 2
  pRecommended.coil.frictionSpeed = 0.0002
  pRecommended.coil.control.forceScale_N = 0.32
  pRecommended.coil.control.integralScale_Ns = 0.02
  pRecommended.coil.control.velocityScale_m_s = 0.1
  pRecommended.coil.control.currentScale_A = 1
  pRecommended.coil.control.surfaceJerkPower = 70
  pRecommended.coil.control.robotJerkPower = 0.2
  pRecommended.coil.control.forceNoise_N = 0.02
  pRecommended.coil.control.strokeNoise_m = 1e-06
  pRecommended.coil.control.frictionPower = 0.0009
  pRecommended.coil.strategy = 'observer'
  pRecommended.coil.forceKp = 0.03
  pRecommended.coil.forceKi = 20
  pRecommended.coil.forceKd = 5e-06
  pRecommended.coil.derivativeFilter = 0.0003
  pRecommended.coil.directCoulombCorrection = 1
  pRecommended.ideal.positionGain = 100
  pRecommended.ideal.velocityTime = 0.005
  pRecommended.ideal.maxSpeed = 0.1
  pRecommended.ideal.maxAcceleration = 20
  pRecommended.ideal.maxAxialForce = Inf
  pRecommended.ideal.forceKp = 7.49999999996e-05
  pRecommended.ideal.forceKi = 0.0179999999999
  pRecommended.ideal.forceKd = 0
  pRecommended.d.M = 1
  pRecommended.d.alpha = 0.4
  pRecommended.d.beta = 0.6
  pRecommended.d.mu = 0.24
  pRecommended.d.g = 9.81
  pRecommended.d.keq = Inf
  pRecommended.d.ell = 0.00159154943092
  pRecommended.d.q10 = 6.266
  pRecommended.d.q20 = -3.544
  pRecommended.d.holdForce = 0.38
  pRecommended.d.r0 = 0
  pRecommended.d.u0 = 0
  pRecommended.d.z0 = 0
  pRecommended.d.forceTicks = 2
  pRecommended.d.sensorTicks = 2
  pRecommended.d.robotTicks = 200
  pRecommended.d.sensorDelaySamples = 1
  pRecommended.d.robotDelaySamples = 8
  pRecommended.d.strokeDelaySamples = 1
  pRecommended.d.duration = 0.1
  pRecommended.d.screwHoldCurrent = 0.012095775675
  pRecommended.d.coilHoldCurrent = 0.019
  pRecommended.d.speedKp = 0.134590250444
  pRecommended.d.speedKi = 40.3770751333
  pRecommended.d.forceKp = 0.03
  pRecommended.d.forceKi = 20
  pRecommended.d.forceFeedforward = 0.019
  pRecommended.d.commandMax = 3.5
  pRecommended.d.commandMin = -3.5
  pRecommended.d.coilControl.A = [0.904837418036  0  0  0  0  0  0  0  0  2.67588421391e-14  -3.29524891735e-09; 0  0.904837418036  0  0  0  0  0  0  0  0  0; 0  0  0.904837418036  0  0  0  0  0  0  0  0; 0  0  0  0.904837418036  0  0  0  0  0  0  0; 0  0  0  0  1  0.01  0  -5e-05  4.99722337924e-05  7.56047730874e-05  0.030764915469; 0  0  0  0  0  1  0  -0.01  0.00999167129437  0.00527845864875  0.0453783132776; 0  0  0  0  0  0  0.367879441171  0  0  -7.29404615433e-13  6.17194806769e-14; 0  0  0  0  0  0  0  1  0  -0.189432576756  0.00157759478786; 0  0  0  0  0  0  0  0  0.998334721451  -2.54541925038e-08  0.00774836045737; 0  0  0  0  0  -0.126424111766  12.6424111766  3.79272335297  0  -0.643457512844  -0.000911475458531; 1  0  0  0  -1  0  0  0  0  -3.22918141347e-05  -0.0303114447317]
  pRecommended.d.coilControl.B = [-2.67588421391e-14  3.29524891735e-06  0  0  0; 0  0  0  0  0; 0  0  0  0  0; 0  0  0  0  0; -7.56047730874e-05  -30.764915469  0  0  5e-06; -0.00527845864875  -45.3783132776  0  0  0.001; 7.29404615433e-13  -6.17194806769e-11  0.632120558829  0  0; 0.189432576756  -1.57759478786  0  0  0; 2.54541925038e-08  -7.74836045737  0  0  0; 1.01133695401  0.911475458531  0  -0.632120558829  0; 3.22918141347e-05  30.3114447317  0  0  0]
  pRecommended.d.coilControl.C = [0.001  0  0  0  0  0  0  0  0  2.95730941335e-17  -3.64181327127e-12; 0  0.1  0  0  0  0  0  0  0  0  0; 0  0  0.001  0  0  0  0  0  0  0  0; 0  0  0  0.1  0  0  0  0  0  0  0; 0  0  0  0  0.001  0  0  0  0  3.22918141643e-08  3.03114410899e-05; 0  0  0  0  0  0.1  0  0  0  0.000338413313594  0.00453165410154; 0  0  0  0  0  0  1  0  0  -1.98272731172e-12  1.67770942786e-13; 0  0  0  0  0  0  0  10  0  -1.89432576756  0.0157759478786; 0  0  0  0  0  0  0  0  10  -2.54966515307e-07  0.0776128515906]
  pRecommended.d.coilControl.D = [-2.95730941335e-17  3.64181327127e-09  0  0  0; 0  0  0  0  0; 0  0  0  0  0; 0  0  0  0  0; -3.22918141643e-08  -0.0303114410899  0  0  0; -0.000338413313594  -4.53165410154  0  0  0; 1.98272731172e-12  -1.67770942786e-10  0  0  0; 1.89432576756  -15.7759478786  0  0  0; 2.54966515307e-07  -77.6128515906  0  0  0]
  pRecommended.d.coilControl.feedback = [0 0 0 0 0 0 -0.584132933117 -0.158413293312 0]
  pRecommended.d.coilControl.integralGain = 1.2641098067
  pRecommended.d.coilControl.force = [0 0 0 0 0 -2 20 2 0]
  pRecommended.d.recenterGain = 0.735294117647
  pRecommended.d.positionMeasurementBias = -0.0125
  pRecommended.d.positionMeasurementInitial = 0.0125
  pRecommended.d.forceKd = 0
  pRecommended.d.derivativeFilter = 0.0003
  pRecommended.springs.maxCombinedLength_m = 0.1
  pRecommended.springs.commonPreload_N = 32
  pRecommended.springs.workingClearance_m = 0.0005
  pRecommended.springs.unseatingClearance_m = 0.00025
  pRecommended.springs.lower.part = 'D-180S'
  pRecommended.springs.lower.rate_N_m = 9873
  pRecommended.springs.lower.freeLength_m = 0.0181
  pRecommended.springs.lower.freeLengthTolerance_m = 0.00049
  pRecommended.springs.lower.minWorkingLength_m = 0.01055
  pRecommended.springs.lower.maxCyclicStroke_m = 0.00318
  pRecommended.springs.lower.forceEnvelope_N = 68.543
  pRecommended.springs.upper.part = 'D-180S'
  pRecommended.springs.upper.rate_N_m = 9873
  pRecommended.springs.upper.freeLength_m = 0.0181
  pRecommended.springs.upper.freeLengthTolerance_m = 0.00049
  pRecommended.springs.upper.minWorkingLength_m = 0.01055
  pRecommended.springs.upper.maxCyclicStroke_m = 0.00318
  pRecommended.springs.upper.forceEnvelope_N = 68.543
  pRecommended.robotPrediction.enabled = 1
  pRecommended.robotPrediction.delay = 0.08
  pRecommended.robotPrediction.responseTime = 0.06
  pRecommended.robotPrediction.maxSpeed = 0.02
  pRecommended.robotPrediction.maxAcceleration = 0.5
  pRecommended.robotPrediction.residualTime = 0.06
  pRecommended.robotPrediction.residualJerkPower = 0.0002
  pRecommended.robotPrediction.boundedNominalPath = 1
  pRecommended.robotPrediction.delaySamples = 8
  pRecommended.robotPrediction.surfaceJerkEnabled = 0
  pRecommended.robotPrediction.surfaceSnapPower = 1000000
  pRecommended.robotPrediction.surfaceJerkDecayTime = Inf
  pRecommended.robotPrediction.surfaceJerkFeedforwardGain = 0
symbols that are objects in the model workspace (value not decoded): p
undefined symbols (not defined in the file or in its folder): DiscIntNeverNeededParam
libraries: sl_discontinuities x1
(part 1 of 4)
settings Model: Creator=tommie  LastModifiedBy=tommie
settings DataIOCC: SignalLogging=off
settings DebuggingCC: AlgebraicLoopMsg=error
settings RTWCC: GenCodeOnly=on
settings GRTTargetCC: MatFileLogging=off

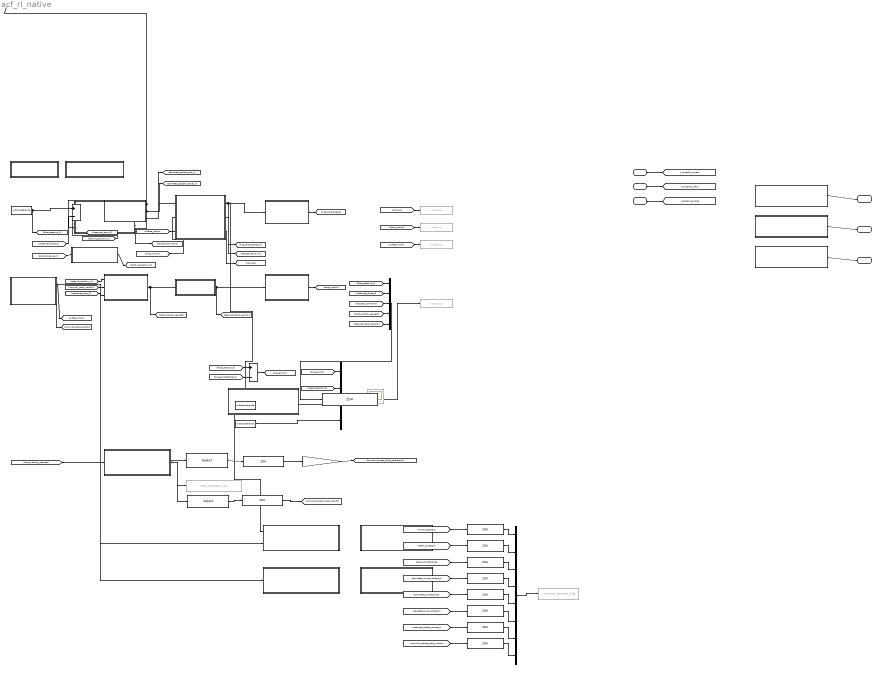
== system acf_rl_native ==
  note: ACTIVE CONTACT FLANGE | native axial model
      | Saved default: voice coil; B+S = 2 kg; 1 mm x 10 mm bump at 100 mm/s.
      | B-S force and S-A relative position; 10 kHz sensing; no known surface preview.
  note: FAST LOOP: true contact force is the performance measure; measured force closes the controller.
  note: SLOW LOOP: flange travel requests robot correction. Delay and motion limits are explicit.
  note: No contact spring/damper. Contact reaction is solved from S motion.
      | The simple model stops at contact loss or a stroke stop and marks the run failed.
  note: Scope order: true error, measured error, +0.5 N, -0.5 N (tolerance is editable).
  note: Double-click Actuator selection to choose Leadscrew or Voice coil.
  note: Named tags carry feedback and logged signals. Click a tag to trace its source.
  rl_current_request_A : Inport  SampleTime=p.force.sampleTime
  rl_robot_correction_m_s : Inport  Port=2  SampleTime=p.force.sampleTime
  rl_baseline_mode : Inport  Port=3  SampleTime=p.force.sampleTime
  ADC acquisition diagnostics : Subsystem
  Actuator and RABS mechanics : Subsystem
  Actuator selection : Subsystem  mask(Active contact flange actuator selection){ActuatorChoice=Voice coil}
      mask prompts: ActuatorChoice "Actuator"
      mask help: Choose the motor before running. Mechanical, surface and sensor settings are preserved. Force-controller gains, command units and initial holding current are recalculated for the selected drive.
      mask TypeOptions ActuatorChoice: Leadscrew | Voice coil | Ideal position (reference)
      mask Callback ActuatorChoice: acf_select_actuator(bdroot(gcb),get_param(gcb,'ActuatorChoice'));
      mask Display: disp(sprintf('Actuator selection\n%s',get_param(gcb,'ActuatorChoice')));
  Command prediction diagnostics : ToWorkspace  Commented=on  VariableName=robot_prediction_log  SaveFormat=Timeseries  SampleTime=p.sim.step
  Contact force measurement : Subsystem
  Control log : ToWorkspace  Commented=on  VariableName=control_log  SaveFormat=Timeseries  SampleTime=p.sim.step
  Control signals : Mux  Inputs=5
  Enable robot acceleration prediction : Gain  Gain=double(p.robotPrediction.enabled)
  Force controller : Subsystem  Variant=on  VariantControlMode=label  LabelModeActiveChoice=Coil PI and PID
  Force controller selection : Subsystem  mask{ControllerChoice=PI, AccelerationFeedforward=on}
      mask prompts: ControllerChoice "Voice-coil control strategy"; AccelerationFeedforward "Measured acceleration feedforward"
      mask help: Native force/stroke observer or conventional force PI/PID. Gains remain editable in the Model Workspace p. The saved recommended preset includes the qualified upper-rigid PID gains.
      mask TypeOptions ControllerChoice: PI | PID
      mask Callback ControllerChoice: acf_select_controller(bdroot);
      mask Callback AccelerationFeedforward: acf_select_controller(bdroot(gcb));
      mask Display: disp('Choose coil controller')
  Force error : Sum  Inputs=+-
  Force error and limits : Mux
  Force measurement : Subsystem
  Force tolerance scope : Scope  Commented=on
  Inertial sensor recordings : Subsystem
  Issued-command robot predictor : Subsystem
  Lateral B-S force measurement : Subsystem
  Lower tolerance : Constant  Value=-p.force.tolerance
  Native control history clock : ZeroOrderHold  SampleTime=p.sim.step
  Normal logging sample {1..8} (8 alike) : ZeroOrderHold  SampleTime=p.sim.step
  Plant log : ToWorkspace  Commented=on  VariableName=plant_log  SaveFormat=Timeseries  SampleTime=p.sim.step
  Predicted robot acceleration : Selector  InputPortWidth=3  IndexOptions=Index vector (dialog)  Indices=3  OutputSizes=1
  Predicted robot velocity : Selector  InputPortWidth=3  IndexOptions=Index vector (dialog)  Indices=2  OutputSizes=1
  Predicted velocity sampling : ZeroOrderHold  SampleTime=p.force.sampleTime
  RL rl_comparator : Subsystem
  RL rl_observation : Subsystem
  RL rl_scoring : Subsystem
  Recenter travel : Subsystem
  Relative position measurement : Subsystem
  Requested force : Constant  Value=p.force.reference
  Robot command delay : Subsystem
  Robot log : ToWorkspace  Commented=on  VariableName=robot_log  SaveFormat=Timeseries  SampleTime=p.sim.step
  Robot motion : Subsystem
  Robot prediction sampling : ZeroOrderHold  SampleTime=p.force.sampleTime
  S accelerometer and ADC : Subsystem
  Surface and nominal path : Subsystem
  Surface contact force : Subsystem
  Surface log : ToWorkspace  Commented=on  VariableName=surface_log  SaveFormat=Timeseries  SampleTime=p.sim.step
  Surface normal diagnostics : Mux  Inputs=8
  Surface normal log : ToWorkspace  Commented=on  VariableName=normal_contact_log  SaveFormat=Timeseries  SampleTime=p.sim.step
  True force error : Sum  Inputs=+-
  Upper tolerance : Constant  Value=p.force.tolerance
  rl_observation : Outport
  rl_scoring : Outport  Port=2
  rl_comparator : Outport  Port=3
  tag scope: command_based_robot_acceleration=global, command_based_robot_velocity=global, estimated_actuator_travel_m=global, estimated_contact_error_N=global, plant_log=global, rl_baseline_mode=global, rl_external_current=global, rl_external_robot=global, surface_motion=global
  wires:
  [robot_motion] -> Actuator and RABS mechanics/2(robot_r_v)
  [surface_motion] -> Actuator and RABS mechanics/3(surface_y_v_a)
  [force_setpoint_N] -> Control signals/1
  [measured_force_N] -> Control signals/2
  [actuator_command] -> Control signals/3
  [robot_velocity_request] -> Control signals/4
  [delayed_robot_velocity] -> Control signals/5
  Force error/1 -> Contact force measurement/1(raw_cell_error_N)
  Requested force/1 -> Force error/1, [force_setpoint_N]
  [measured_force_N] -> Force error/2
  [true_error_N] -> Force error and limits/1
  [measured_error_N] -> Force error and limits/2
  Upper tolerance/1 -> Force error and limits/3
  Lower tolerance/1 -> Force error and limits/4
  Actuator and RABS mechanics/1(true_Fc_N) -> Force measurement/1(true_Fc_N), [true_contact_force_N], Surface contact force/1(Axial reaction)
  Force error and limits/1 -> Force tolerance scope/1
  [plant_log] -> Plant log/1
  [relative_position_m] -> Recenter travel/1(travel_m)
  [nominal_robot_velocity] -> Recenter travel/2(nominal_velocity)
  Recenter travel/1(requested_velocity) -> Robot command delay/1(requested_velocity), [robot_velocity_request]
  [robot_motion] -> Robot log/1
  Robot command delay/1(delayed_velocity) -> Robot motion/1(delayed_velocity), [delayed_robot_velocity]
  Actuator and RABS mechanics/2(travel_m) -> [actuator_travel_m]
  Force measurement/1(measured_Fc_N) -> [measured_force_N]
  Surface and nominal path/2(nominal_velocity) -> [nominal_robot_velocity]
  Actuator and RABS mechanics/3(diagnostics) -> [plant_log]
  Robot motion/1(actual_r_v) -> [robot_motion]
  Surface and nominal path/1(surface_y_v_a) -> [surface_motion], Surface contact force/2(Physical surface velocity), S accelerometer and ADC/1(Physical S motion)
  True force error/1 -> [true_error_N]
  [surface_motion] -> Surface log/1
  [force_setpoint_N] -> True force error/1
  [true_contact_force_N] -> True force error/2
  [actuator_travel_m] -> Relative position measurement/1(travel_m)
  Relative position measurement/1(measured_travel_m) -> [relative_position_m]
  Force controller/1(command) -> Actuator and RABS mechanics/1(command), [actuator_command], Contact force measurement/3(Issued selected actuator request)
  [measured_error_N] -> Recenter travel/3(measured_force_error_N)
  Force controller/2(estimated_travel_m) -> [estimated_actuator_travel_m]
  Force controller/3(estimated_force_error_N) -> [estimated_contact_error_N]
  [robot_velocity_request] -> Issued-command robot predictor/1(issued_velocity_request)
  Issued-command robot predictor/1(predicted_r_v_a) -> Predicted robot acceleration/1, Command prediction diagnostics/1, Predicted robot velocity/1
  Predicted robot acceleration/1 -> Robot prediction sampling/1
  Robot prediction sampling/1 -> Enable robot acceleration prediction/1
  Enable robot acceleration prediction/1 -> [command_based_robot_acceleration]
  Predicted robot velocity/1 -> Predicted velocity sampling/1
  Predicted velocity sampling/1 -> [command_based_robot_velocity]
  [normal_contact_N] -> Normal logging sample 1/1
  Normal logging sample 1/1 -> Surface normal diagnostics/1
  [lateral_contact_N] -> Normal logging sample 2/1
  Normal logging sample 2/1 -> Surface normal diagnostics/2
  [actual_contact_slope] -> Normal logging sample 3/1
  Normal logging sample 3/1 -> Surface normal diagnostics/3
  [estimated_normal_contact_N] -> Normal logging sample 4/1
  Normal logging sample 4/1 -> Surface normal diagnostics/4
  [estimated_contact_slope] -> Normal logging sample 5/1
  Normal logging sample 5/1 -> Surface normal diagnostics/5
  [requested_axial_contact_N] -> Normal logging sample 6/1
  Normal logging sample 6/1 -> Surface normal diagnostics/6
  [measured_lateral_contact_N] -> Normal logging sample 7/1
  Normal logging sample 7/1 -> Surface normal diagnostics/7
  [command_based_robot_velocity] -> Normal logging sample 8/1
  Normal logging sample 8/1 -> Surface normal diagnostics/8
  Surface normal diagnostics/1 -> Surface normal log/1
  [relative_position_m] -> Contact force measurement/2(measured_head_position_m)
  Contact force measurement/1(normal_force_error_N) -> Force controller/1(error_N), [measured_error_N]
  Contact force measurement/2(estimated_head_travel_m) -> Force controller/2(measured_travel_m)
  Control signals/1 -> Native control history clock/1
  Native control history clock/1 -> Control log/1
  rl_current_request_A/1 -> [rl_external_current]
  rl_robot_correction_m_s/1 -> [rl_external_robot]
  rl_baseline_mode/1 -> [rl_baseline_mode]
  RL rl_observation/1(output) -> rl_observation/1
  RL rl_scoring/1(output) -> rl_scoring/1
  RL rl_comparator/1(output) -> rl_comparator/1

== system acf_rl_native/ADC acquisition diagnostics ==
  ADC native conversion channels : Mux  Inputs=8
  All ADC conversion samples : ToWorkspace  Commented=on  VariableName=adc_acquisition_log  SaveFormat=Timeseries  SampleTime=p.adcStudy.outputSampleTime_s
  wires:
  [force_adc_prequant] -> ADC native conversion channels/1
  [lateral_adc_prequant] -> ADC native conversion channels/2
  [acceleration_z_adc_prequant] -> ADC native conversion channels/3
  [acceleration_x_adc_prequant] -> ADC native conversion channels/4
  [force_adc_clip] -> ADC native conversion channels/5
  [lateral_adc_clip] -> ADC native conversion channels/6
  [acceleration_z_adc_clip] -> ADC native conversion channels/7
  [acceleration_x_adc_clip] -> ADC native conversion channels/8
  ADC native conversion channels/1 -> All ADC conversion samples/1

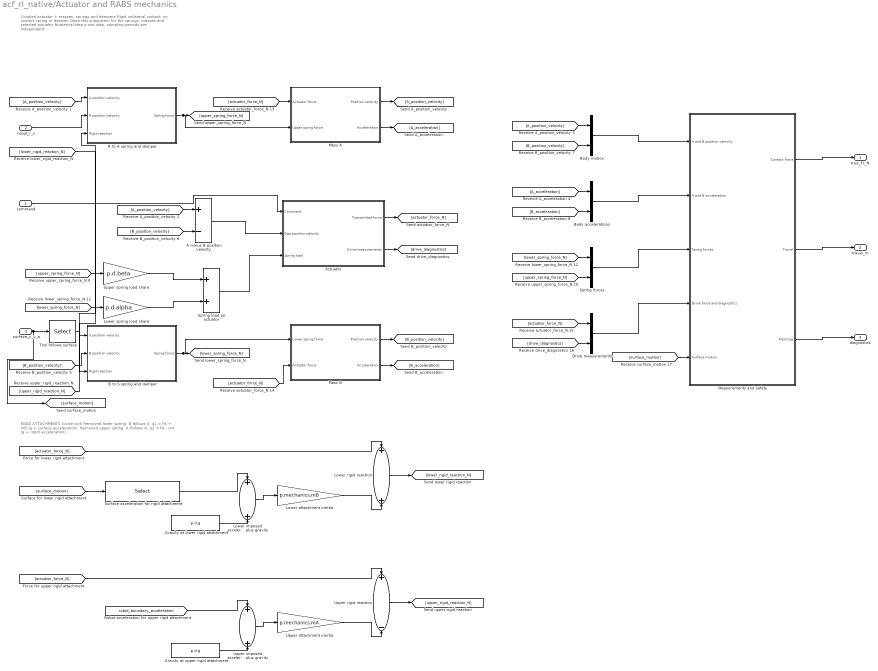
== system acf_rl_native/Actuator and RABS mechanics ==
  note: Coupled actuator + masses, springs and dampers
      | Rigid unilateral contact; no contact spring or damper
      | Open this subsystem for the springs, masses and selected actuator
      | Numerical step p.sim.step; sampling periods are independent.
  note: RIGID ATTACHMENTS (voice coil)
      | Removed lower spring: B follows S, q1 = Fa + mB (g + surface acceleration).
      | Removed upper spring: A follows R, q2 = Fa - mA (g + robot acceleration).
  command : Inport
  robot_r_v : Inport  Port=2
  surface_y_v_a : Inport  Port=3
  A minus B position velocity : Sum  Inputs=+-
  Actuator : Subsystem  Variant=on  VariantControlMode=label  LabelModeActiveChoice=Voice coil
  B to S spring and damper : Subsystem
  Body accelerations : Mux  Inputs=2
  Body motion : Mux  Inputs=2
  Drive measurements : Mux  Inputs=2
  Gravity at lower rigid attachment : Constant  Value=p.d.g
  Gravity at upper rigid attachment : Constant  Value=p.d.g
  Lower attachment inertia : Gain  Gain=p.mechanics.mB
  Lower imposed acceleration plus gravity : Sum
  Lower rigid reaction : Sum
  Lower spring load share : Gain  Gain=p.d.alpha
  Mass A : Subsystem
  Mass B : Subsystem
  Measurements and safety : Subsystem
  R to A spring and damper : Subsystem
  Spring forces : Mux  Inputs=2
  Spring load on actuator : Sum
  Surface acceleration for rigid attachment : Selector  InputPortWidth=3  IndexOptions=Index vector (dialog)  Indices=3  OutputSizes=1
  Tool follows surface : Selector  InputPortWidth=3  IndexOptions=Index vector (dialog)  Indices=[1 2]  OutputSizes=1
  Upper attachment inertia : Gain  Gain=p.mechanics.mA
  Upper imposed acceleration plus gravity : Sum
  Upper rigid reaction : Sum  Inputs=+-
  Upper spring load share : Gain  Gain=p.d.beta
  true_Fc_N : Outport
  travel_m : Outport  Port=2
  diagnostics : Outport  Port=3
  wires:
  [A_position_velocity] -> A minus B position velocity/1
  [B_position_velocity] -> A minus B position velocity/2
  command/1 -> Actuator/1(Command)
  A minus B position velocity/1 -> Actuator/2(Gap position velocity)
  Spring load on actuator/1 -> Actuator/3(Spring load)
  Tool follows surface/1 -> B to S spring and damper/1(S position velocity)
  [B_position_velocity] -> B to S spring and damper/2(B position velocity)
  [A_acceleration] -> Body accelerations/1
  [B_acceleration] -> Body accelerations/2
  [A_position_velocity] -> Body motion/1
  [B_position_velocity] -> Body motion/2
  [actuator_force_N] -> Drive measurements/1
  [drive_diagnostics] -> Drive measurements/2
  [lower_spring_force_N] -> Lower spring load share/1
  [actuator_force_N] -> Mass A/1(Actuator force)
  R to A spring and damper/1(Spring force) -> Mass A/2(Upper spring force), [upper_spring_force_N]
  B to S spring and damper/1(Spring force) -> Mass B/1(Lower spring force), [lower_spring_force_N]
  [actuator_force_N] -> Mass B/2(Actuator force)
  Body motion/1 -> Measurements and safety/1(A and B position velocity)
  Body accelerations/1 -> Measurements and safety/2(A and B acceleration)
  Spring forces/1 -> Measurements and safety/3(Spring forces)
  Drive measurements/1 -> Measurements and safety/4(Drive force and diagnostics)
  [surface_motion] -> Measurements and safety/5(Surface motion)
  [A_position_velocity] -> R to A spring and damper/1(A position velocity)
  robot_r_v/1 -> R to A spring and damper/2(R position velocity)
  Mass A/2(Acceleration) -> [A_acceleration]
  Mass A/1(Position velocity) -> [A_position_velocity]
  Mass B/2(Acceleration) -> [B_acceleration]
  Mass B/1(Position velocity) -> [B_position_velocity]
  Actuator/1(Transmitted force) -> [actuator_force_N]
  Actuator/2(Drive measurements) -> [drive_diagnostics]
  surface_y_v_a/1 -> [surface_motion], Tool follows surface/1
  [lower_spring_force_N] -> Spring forces/1
  [upper_spring_force_N] -> Spring forces/2
  Upper spring load share/1 -> Spring load on actuator/1
  Lower spring load share/1 -> Spring load on actuator/2
  [upper_spring_force_N] -> Upper spring load share/1
  Measurements and safety/1(Contact force) -> true_Fc_N/1
  Measurements and safety/2(Travel) -> travel_m/1
  Measurements and safety/3(Plant log) -> diagnostics/1
  [actuator_force_N] -> Lower rigid reaction/1
  [surface_motion] -> Surface acceleration for rigid attachment/1
  Surface acceleration for rigid attachment/1 -> Lower imposed acceleration plus gravity/1
  Gravity at lower rigid attachment/1 -> Lower imposed acceleration plus gravity/2
  Lower imposed acceleration plus gravity/1 -> Lower attachment inertia/1
  Lower attachment inertia/1 -> Lower rigid reaction/2
  Lower rigid reaction/1 -> [lower_rigid_reaction_N]
  [actuator_force_N] -> Upper rigid reaction/1
  [robot_boundary_acceleration] -> Upper imposed acceleration plus gravity/1
  Gravity at upper rigid attachment/1 -> Upper imposed acceleration plus gravity/2
  Upper imposed acceleration plus gravity/1 -> Upper attachment inertia/1
  Upper attachment inertia/1 -> Upper rigid reaction/2
  Upper rigid reaction/1 -> [upper_rigid_reaction_N]
  [lower_rigid_reaction_N] -> B to S spring and damper/3(Rigid reaction)
  [upper_rigid_reaction_N] -> R to A spring and damper/3(Rigid reaction)

== system acf_rl_native/Actuator selection ==

== system acf_rl_native/Contact force measurement ==
  raw_cell_error_N : Inport
  measured_head_position_m : Inport  Port=2
  Issued selected actuator request : Inport  Port=3
  Contact force reconstruction : Subsystem
  Head motion estimator : Subsystem
  Normal force error sign : Gain  Gain=-1
  Normal force projection : Subsystem
  normal_force_error_N : Outport
  estimated_head_travel_m : Outport  Port=2
  tag scope: inertial_axial_reference_deviation_N=global, inertial_head_gap_velocity=global
  wires:
  raw_cell_error_N/1 -> Contact force reconstruction/1(raw_cell_error_N)
  measured_head_position_m/1 -> Head motion estimator/1(measured_head_position_m)
  Contact force reconstruction/1(axial_contact_N) -> Normal force projection/1(Compensated axial force)
  Contact force reconstruction/2(lateral_contact_N) -> Normal force projection/2(Compensated lateral force)
  Head motion estimator/1(head_gap_velocity_m_s) -> Normal force projection/3(Head gap velocity), [inertial_head_gap_velocity]
  Head motion estimator/2(estimated_head_travel_m) -> estimated_head_travel_m/1
  Normal force projection/1(normal_force_deviation_N) -> Normal force error sign/1
  Normal force error sign/1 -> normal_force_error_N/1
  Normal force projection/2(axial_reference_deviation_N) -> [inertial_axial_reference_deviation_N]
  Issued selected actuator request/1 -> Head motion estimator/2(Issued post-limit current request)

== system acf_rl_native/Force controller ==
  error_N : Inport
  measured_travel_m : Inport  Port=2
  Coil PI and PID : Subsystem  VariantControl=Coil PI and PID
  Drive PI and PID : Subsystem  VariantControl=Drive PI and PID
  command : Outport
  estimated_travel_m : Outport  Port=2
  estimated_force_error_N : Outport  Port=3

== system acf_rl_native/Force controller selection ==

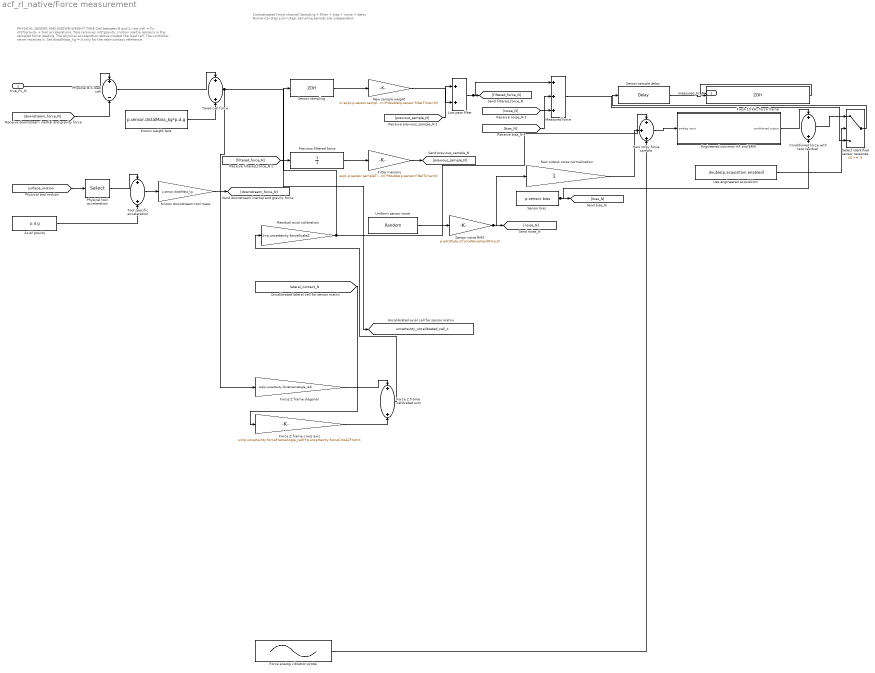
== system acf_rl_native/Force measurement ==
  note: Compensated force channel
      | Sampling + filter + bias + noise + delay
      | Numerical step p.sim.step; sampling periods are independent.
  note: PHYSICAL SENSOR AND KNOWN-WEIGHT TARE
      | Cell between B and S: raw cell = Fc - mS*(gravity + tool acceleration).
      | Tare removes mS*gravity; motion inertia remains in the sampled force reading.
      | The physical acceleration above models the load cell. The controller never receives it.
      | Set distalMass_kg = 0 only for the near-contact reference.
  true_Fc_N : Inport
  Axial gravity : Constant  Value=p.d.g
  Conditioned force with tare residual : Sum
  Engineered common AA and EMA : Subsystem
  Filter memory : Gain  Gain=exp(-p.sensor.sampleTime/max(p.sensor.filterTime,realmin))*double(p.sensor.filterTime>0)
  Force Z frame calibrated sum : Sum
  Force Z frame cross axis : Gain  Gain=sin(p.uncertainty.forceFrameAngle_rad)+p.uncertainty.forceCrossZFromX
  Force Z frame diagonal : Gain  Gain=cos(p.uncertainty.forceFrameAngle_rad)
  Force analog vibration probe : Sin  Amplitude=p.adcStudy.forceAnalogToneAmplitude_N  Frequency=2*pi*p.adcStudy.analogToneFrequency_Hz  Phase=p.adcStudy.analogTonePhase_rad  SampleTime=0
  Fresh 10 kHz force frame : ZeroOrderHold  SampleTime=p.force.sampleTime
  Known downstream tool mass : Gain  Gain=p.sensor.distalMass_kg
  Known weight tare : Constant  Value=p.sensor.distalMass_kg*p.d.g
  Low pass filter : Sum
  Measured force : Sum  Inputs=+++
  New sample weight : Gain  Gain=1-(exp(-p.sensor.sampleTime/max(p.sensor.filterTime,realmin))*double(p.sensor.filterTime>0))
  Physical B-S load cell : Sum  Inputs=+-
  Physical tool acceleration : Selector  InputPortWidth=3  IndexOptions=Index vector (dialog)  Indices=3  OutputSizes=1
  Previous filtered force : UnitDelay  InitialCondition=p.force.reference*(1+p.uncertainty.forceScaleZ)*(cos(p.uncertainty.forceFrameAngle_rad)-p.contact.mu*(sin(p.uncertainty.forceFrameAngle_rad)+p.uncertainty.forceCrossZFromX))  SampleTime=p.sensor.sampleTime
  Raw noisy force sample : Sum  Inputs=+++
  Raw output-noise normalization : Gain
  Residual axial calibration : Gain  Gain=1+p.uncertainty.forceScaleZ
  Select identified sensor response : Switch  Threshold=.5  SaturateOnIntegerOverflow=off  InputSameDT=off
  Sensor bias : Constant  Value=p.sensor.bias
  Sensor noise RMS : Gain  Gain=p.adcStudy.d.forceNoiseInputRms_N
  Sensor sample delay : TransportDelay  DelayTime=p.adcStudy.d.channels.force.pipelineDelay_s  InitialOutput=round((((p.force.reference*(1+p.uncertainty.forceScaleZ)*(cos(p.uncertainty.forceFrameAngle_rad)-p.contact.mu*(sin(p.uncertainty.forceFrameAngle_rad)+p.uncertainty.forceCrossZFromX))))+(p.adcStudy.d.forceGravityOffset_N))/(max(p.adcStudy.forceQuantum_N,1e-15)))*(max(p.adcStudy.forceQuantum_N,1e-15))-round((p.adcStudy.d.forceGravityOffset_N)/(max(p.adcStudy.forceQuantum_N,1e-15)))*(max(p.adcStudy.forceQuantum_N,1e-15))+(p.sensor.bias)
  Sensor sampling : ZeroOrderHold  SampleTime=p.sensor.sampleTime
  Tared cell force : Sum
  Tool specific acceleration : Sum
  Uniform sensor noise : UniformRandomNumber  Minimum=-sqrt(3)  Maximum=sqrt(3)  Seed=p.sensor.seed  SampleTime=p.sensor.sampleTime
  Use engineered acquisition : Constant  Value=double(p.acquisition.enabled)
  measured_Fc_N : Outport
  tag scope: uncertainty_uncalibrated_cell_z=global
  wires:
  Previous filtered force/1 -> Filter memory/1
  [previous_sample_N] -> Low pass filter/1
  New sample weight/1 -> Low pass filter/2
  Low pass filter/1 -> Measured force/1, [filtered_force_N]
  [bias_N] -> Measured force/2
  [noise_N] -> Measured force/3
  Sensor sampling/1 -> New sample weight/1
  [filtered_force_N] -> Previous filtered force/1
  Sensor bias/1 -> [bias_N], Conditioned force with tare residual/2
  Sensor noise RMS/1 -> [noise_N], Raw output-noise normalization/1
  Filter memory/1 -> [previous_sample_N]
  Uniform sensor noise/1 -> Sensor noise RMS/1
  Measured force/1 -> Select identified sensor response/3
  true_Fc_N/1 -> Physical B-S load cell/1
  [downstream_force_N] -> Physical B-S load cell/2
  Physical B-S load cell/1 -> Tared cell force/1
  Known weight tare/1 -> Tared cell force/2
  [surface_motion] -> Physical tool acceleration/1
  Physical tool acceleration/1 -> Tool specific acceleration/1
  Axial gravity/1 -> Tool specific acceleration/2
  Tool specific acceleration/1 -> Known downstream tool mass/1
  Known downstream tool mass/1 -> [downstream_force_N]
  Raw output-noise normalization/1 -> Raw noisy force sample/2
  Conditioned force with tare residual/1 -> Select identified sensor response/1
  Use engineered acquisition/1 -> Select identified sensor response/2
  Fresh 10 kHz force frame/1 -> measured_Fc_N/1
  Tared cell force/1 -> [uncertainty_uncalibrated_cell_z], Force Z frame diagonal/1
  Residual axial calibration/1 -> Sensor sampling/1, Raw noisy force sample/1
  [lateral_contact_N] -> Force Z frame cross axis/1
  Force Z frame diagonal/1 -> Force Z frame calibrated sum/1
  Force Z frame cross axis/1 -> Force Z frame calibrated sum/2
  Force Z frame calibrated sum/1 -> Residual axial calibration/1
  Force analog vibration probe/1 -> Raw noisy force sample/3
  Raw noisy force sample/1 -> Engineered common AA and EMA/1(analog input)
  Engineered common AA and EMA/1(conditioned output) -> Conditioned force with tare residual/1
  Select identified sensor response/1 -> Sensor sample delay/1
  Sensor sample delay/1 -> Fresh 10 kHz force frame/1

== system acf_rl_native/Inertial sensor recordings ==
  Acceleration and reconstructed force : Mux  Inputs=6
  Acceleration validation log : ToWorkspace  Commented=on  VariableName=accelerometer_log  SaveFormat=Timeseries  SampleTime=p.sim.step
  Head motion recording clock : ZeroOrderHold  SampleTime=p.sim.step
  Motion observer validation log : ToWorkspace  Commented=on  VariableName=inertial_motion_log  SaveFormat=Timeseries  SampleTime=p.sim.step
  Record every physical step {1..6} (6 alike) : ZeroOrderHold  SampleTime=p.sim.step
  wires:
  [measured_S_acceleration_z] -> Record every physical step 1/1
  Record every physical step 1/1 -> Acceleration and reconstructed force/1
  [measured_S_acceleration_x] -> Record every physical step 2/1
  Record every physical step 2/1 -> Acceleration and reconstructed force/2
  [physical_S_acceleration_z] -> Record every physical step 3/1
  Record every physical step 3/1 -> Acceleration and reconstructed force/3
  [physical_S_acceleration_x] -> Record every physical step 4/1
  Record every physical step 4/1 -> Acceleration and reconstructed force/4
  [inertial_axial_contact_N] -> Record every physical step 5/1
  Record every physical step 5/1 -> Acceleration and reconstructed force/5
  [inertial_lateral_contact_N] -> Record every physical step 6/1
  Record every physical step 6/1 -> Acceleration and reconstructed force/6
  Acceleration and reconstructed force/1 -> Acceleration validation log/1
  [inertial_head_motion_states] -> Head motion recording clock/1
  Head motion recording clock/1 -> Motion observer validation log/1

== system acf_rl_native/Issued-command robot predictor ==
  issued_velocity_request : Inport
  Expected acceleration limit : Saturate  UpperLimit=p.robotPrediction.maxAcceleration  LowerLimit=-p.robotPrediction.maxAcceleration
  Expected command delay : Delay  DelayLengthSource=Input port  DelayLength=p.robotPrediction.delaySamples  DelayLengthUpperLimit=12  InitialCondition=p.robot.nominalVelocity*double(~p.robotPrediction.boundedNominalPath)  PreventDirectFeedthrough=on  DiagnosticForDelayLength=Error  UseCircularBuffer=on  SampleTime=p.robot.sampleTime
      settings: InputPortMap=u0,p1
  Expected speed limit : Saturate  UpperLimit=p.robotPrediction.maxSpeed  LowerLimit=-p.robotPrediction.maxSpeed
  Expected velocity response : Gain  Gain=1/p.robotPrediction.responseTime
  Predicted position velocity acceleration : Mux  Inputs=3
  Predicted relative position : Integrator
  Predicted velocity : Integrator
  Predicted velocity error : Sum  Inputs=+-
  RL reset-fixed queue length : Constant  Value=p.robotPrediction.delaySamples
  predicted_r_v_a : Outport
  wires:
  Predicted position velocity acceleration/1 -> predicted_r_v_a/1
  Predicted relative position/1 -> Predicted position velocity acceleration/1
  Predicted velocity/1 -> Predicted position velocity acceleration/2, Predicted relative position/1, [prediction_internal_velocity]
  Expected acceleration limit/1 -> Predicted position velocity acceleration/3, Predicted velocity/1
  Expected velocity response/1 -> Expected acceleration limit/1
  Predicted velocity error/1 -> Expected velocity response/1
  [prediction_internal_velocity] -> Predicted velocity error/2
  Expected speed limit/1 -> Predicted velocity error/1
  Expected command delay/1 -> Expected speed limit/1
  issued_velocity_request/1 -> Expected command delay/1
  RL reset-fixed queue length/1 -> Expected command delay/2

== system acf_rl_native/Lateral B-S force measurement ==
  Conditioned force with tare residual : Sum
  Engineered common AA and EMA : Subsystem
  Filter memory : UnitDelay  InitialCondition=p.force.reference*(1+p.uncertainty.forceScaleX)*(-p.contact.mu*cos(p.uncertainty.forceFrameAngle_rad)-sin(p.uncertainty.forceFrameAngle_rad)+p.uncertainty.forceCrossXFromZ)  SampleTime=p.sensor.sampleTime
  Filtered derivative memory : Gain  Gain=exp(-p.sensor.sampleTime/p.contact.lateralDerivativeFilterTime_s)
  Filtered derivative new sample : Gain  Gain=(1-exp(-p.sensor.sampleTime/p.contact.lateralDerivativeFilterTime_s))/p.sensor.sampleTime
  Filtered lateral force derivative : Sum
  Force X frame calibrated sum : Sum
  Force X frame cross axis : Gain  Gain=-sin(p.uncertainty.forceFrameAngle_rad)+p.uncertainty.forceCrossXFromZ
  Force X frame diagonal : Gain  Gain=cos(p.uncertainty.forceFrameAngle_rad)
  Fresh 10 kHz force frame : ZeroOrderHold  SampleTime=p.force.sampleTime
  Identified lateral latency : Gain  Gain=p.contact.lateralPredictionTime_s
  Independent lateral noise : UniformRandomNumber  Minimum=-sqrt(3)  Maximum=sqrt(3)  Seed=p.sensor.seed+197  SampleTime=p.sensor.sampleTime
  Known tare residual bias : Constant  Value=p.contact.lateralBias_N
  Lateral analog vibration probe : Sin  Amplitude=p.adcStudy.lateralAnalogToneAmplitude_N  Frequency=2*pi*p.adcStudy.analogToneFrequency_Hz  Phase=p.adcStudy.analogTonePhase_rad  SampleTime=0
  Measured lateral force increment : Sum  Inputs=+-
  New sample weight : Gain  Gain=1-exp(-p.sensor.sampleTime/max(p.sensor.filterTime,realmin))*double(p.sensor.filterTime>0)
  Noise RMS : Gain  Gain=p.adcStudy.d.lateralNoiseInputRms_N
  Noisy tared lateral force : Sum  Inputs=+++
  Old sample weight : Gain  Gain=exp(-p.sensor.sampleTime/max(p.sensor.filterTime,realmin))*double(p.sensor.filterTime>0)
  Present lateral force estimate : Sum
  Previous lateral derivative : UnitDelay  SampleTime=p.sensor.sampleTime
  Previous measured lateral force : UnitDelay  InitialCondition=p.force.reference*(1+p.uncertainty.forceScaleX)*(-p.contact.mu*cos(p.uncertainty.forceFrameAngle_rad)-sin(p.uncertainty.forceFrameAngle_rad)+p.uncertainty.forceCrossXFromZ)+p.contact.lateralBias_N  SampleTime=p.sensor.sampleTime
  Raw noisy force sample : Sum  Inputs=+++
  Raw output-noise normalization : Gain
  Residual lateral calibration : Gain  Gain=1+p.uncertainty.forceScaleX
  Select identified sensor response : Switch  Threshold=.5  SaturateOnIntegerOverflow=off  InputSameDT=off
  Sensor low pass : Sum
  Sensor sample delay : TransportDelay  DelayTime=p.adcStudy.d.channels.lateral.pipelineDelay_s  InitialOutput=round((((p.force.reference*(1+p.uncertainty.forceScaleX)*(-p.contact.mu*cos(p.uncertainty.forceFrameAngle_rad)-sin(p.uncertainty.forceFrameAngle_rad)+p.uncertainty.forceCrossXFromZ)))+(p.adcStudy.d.lateralGravityOffset_N))/(max(p.adcStudy.forceQuantum_N,1e-15)))*(max(p.adcStudy.forceQuantum_N,1e-15))-round((p.adcStudy.d.lateralGravityOffset_N)/(max(p.adcStudy.forceQuantum_N,1e-15)))*(max(p.adcStudy.forceQuantum_N,1e-15))+(p.contact.lateralBias_N)
  Sensor sampling : ZeroOrderHold  SampleTime=p.sensor.sampleTime
  Use engineered acquisition : Constant  Value=double(p.acquisition.enabled)
  tag scope: measured_lateral_contact_N=global, predicted_lateral_contact_N=global
  wires:
  Sensor sampling/1 -> New sample weight/1
  New sample weight/1 -> Sensor low pass/1
  Sensor low pass/1 -> Filter memory/1, Noisy tared lateral force/1
  Filter memory/1 -> Old sample weight/1
  Old sample weight/1 -> [normal_lateral_filter_local]
  [normal_lateral_filter_local] -> Sensor low pass/2
  Independent lateral noise/1 -> Noise RMS/1
  Noise RMS/1 -> Noisy tared lateral force/2, Raw output-noise normalization/1
  Known tare residual bias/1 -> Noisy tared lateral force/3, Conditioned force with tare residual/2
  Noisy tared lateral force/1 -> Select identified sensor response/3
  Previous measured lateral force/1 -> Measured lateral force increment/2
  Measured lateral force increment/1 -> Filtered derivative new sample/1
  Filtered derivative new sample/1 -> Filtered lateral force derivative/1
  Filtered lateral force derivative/1 -> Previous lateral derivative/1, Identified lateral latency/1
  Previous lateral derivative/1 -> Filtered derivative memory/1
  Filtered derivative memory/1 -> Filtered lateral force derivative/2
  Identified lateral latency/1 -> Present lateral force estimate/2
  Present lateral force estimate/1 -> [predicted_lateral_contact_N]
  Raw output-noise normalization/1 -> Raw noisy force sample/2
  Conditioned force with tare residual/1 -> Select identified sensor response/1
  Use engineered acquisition/1 -> Select identified sensor response/2
  Fresh 10 kHz force frame/1 -> [measured_lateral_contact_N], Previous measured lateral force/1, Measured lateral force increment/1, Present lateral force estimate/1
  Residual lateral calibration/1 -> Sensor sampling/1, Raw noisy force sample/1
  [lateral_contact_N] -> Force X frame diagonal/1
  [uncertainty_uncalibrated_cell_z] -> Force X frame cross axis/1
  Force X frame diagonal/1 -> Force X frame calibrated sum/1
  Force X frame cross axis/1 -> Force X frame calibrated sum/2
  Force X frame calibrated sum/1 -> Residual lateral calibration/1
  Lateral analog vibration probe/1 -> Raw noisy force sample/3
  Raw noisy force sample/1 -> Engineered common AA and EMA/1(analog input)
  Engineered common AA and EMA/1(conditioned output) -> Conditioned force with tare residual/1
  Select identified sensor response/1 -> Sensor sample delay/1
  Sensor sample delay/1 -> Fresh 10 kHz force frame/1

== system acf_rl_native/RL rl_comparator ==
  Double 1 : DataTypeConversion  OutDataTypeStr=double  SaturateOnIntegerOverflow=off  RndMeth=Floor
  Double 2 : DataTypeConversion  OutDataTypeStr=double  SaturateOnIntegerOverflow=off  RndMeth=Floor
  Double 3 : DataTypeConversion  OutDataTypeStr=double  SaturateOnIntegerOverflow=off  RndMeth=Floor
  Vector : Mux  Inputs=3
  output : Outport
  wires:
  [rl_baseline_current] -> Double 1/1
  Double 1/1 -> Vector/1
  [rl_baseline_robot] -> Double 2/1
  Double 2/1 -> Vector/2
  [rl_equilibrium_current] -> Double 3/1
  Double 3/1 -> Vector/3
  Vector/1 -> output/1

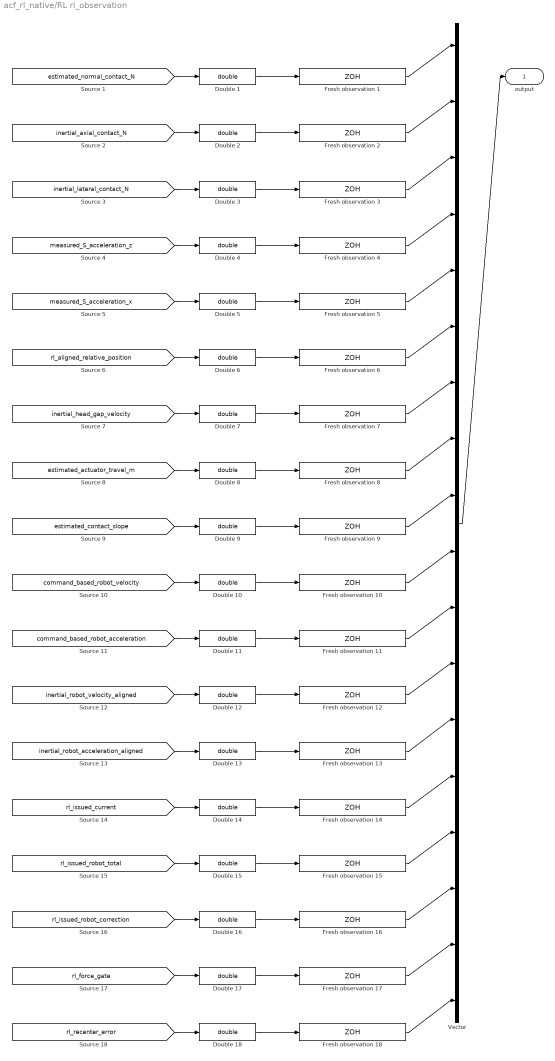
== system acf_rl_native/RL rl_observation ==
  Double {1..18} (18 alike) : DataTypeConversion  OutDataTypeStr=double  SaturateOnIntegerOverflow=off  RndMeth=Floor
  Fresh observation {1..18} (18 alike) : ZeroOrderHold  SampleTime=p.force.sampleTime
  Vector : Mux  Inputs=18
  output : Outport
  wires:
  [estimated_normal_contact_N] -> Double 1/1
  Double 1/1 -> Fresh observation 1/1
  Fresh observation 1/1 -> Vector/1
  [inertial_axial_contact_N] -> Double 2/1
  Double 2/1 -> Fresh observation 2/1
  Fresh observation 2/1 -> Vector/2
  [inertial_lateral_contact_N] -> Double 3/1
  Double 3/1 -> Fresh observation 3/1
  Fresh observation 3/1 -> Vector/3
  [measured_S_acceleration_z] -> Double 4/1
  Double 4/1 -> Fresh observation 4/1
  Fresh observation 4/1 -> Vector/4
  [measured_S_acceleration_x] -> Double 5/1
  Double 5/1 -> Fresh observation 5/1
  Fresh observation 5/1 -> Vector/5
  [rl_aligned_relative_position] -> Double 6/1
  Double 6/1 -> Fresh observation 6/1
  Fresh observation 6/1 -> Vector/6
  [inertial_head_gap_velocity] -> Double 7/1
  Double 7/1 -> Fresh observation 7/1
  Fresh observation 7/1 -> Vector/7
  [estimated_actuator_travel_m] -> Double 8/1
  Double 8/1 -> Fresh observation 8/1
  Fresh observation 8/1 -> Vector/8
  [estimated_contact_slope] -> Double 9/1
  Double 9/1 -> Fresh observation 9/1
  Fresh observation 9/1 -> Vector/9
  [command_based_robot_velocity] -> Double 10/1
  Double 10/1 -> Fresh observation 10/1
  Fresh observation 10/1 -> Vector/10
  [command_based_robot_acceleration] -> Double 11/1
  Double 11/1 -> Fresh observation 11/1
  Fresh observation 11/1 -> Vector/11
  [inertial_robot_velocity_aligned] -> Double 12/1
  Double 12/1 -> Fresh observation 12/1
  Fresh observation 12/1 -> Vector/12
  [inertial_robot_acceleration_aligned] -> Double 13/1
  Double 13/1 -> Fresh observation 13/1
  Fresh observation 13/1 -> Vector/13
  [rl_issued_current] -> Double 14/1
  Double 14/1 -> Fresh observation 14/1
  Fresh observation 14/1 -> Vector/14
  [rl_issued_robot_total] -> Double 15/1
  Double 15/1 -> Fresh observation 15/1
  Fresh observation 15/1 -> Vector/15
  [rl_issued_robot_correction] -> Double 16/1
  Double 16/1 -> Fresh observation 16/1
  Fresh observation 16/1 -> Vector/16
  [rl_force_gate] -> Double 17/1
  Double 17/1 -> Fresh observation 17/1
  Fresh observation 17/1 -> Vector/17
  [rl_recenter_error] -> Double 18/1
  Double 18/1 -> Fresh observation 18/1
  Fresh observation 18/1 -> Vector/18
  Vector/1 -> output/1

== system acf_rl_native/RL rl_scoring ==
  Double 1 : DataTypeConversion  OutDataTypeStr=double  SaturateOnIntegerOverflow=off  RndMeth=Floor
  Double 2 : DataTypeConversion  OutDataTypeStr=double  SaturateOnIntegerOverflow=off  RndMeth=Floor
  Double 3 : DataTypeConversion  OutDataTypeStr=double  SaturateOnIntegerOverflow=off  RndMeth=Floor
  Vector : Mux  Inputs=3
  output : Outport
  wires:
  [normal_contact_N] -> Double 1/1
  Double 1/1 -> Vector/1
  [plant_log] -> Double 2/1
  Double 2/1 -> Vector/2
  [actual_contact_slope] -> Double 3/1
  Double 3/1 -> Vector/3
  Vector/1 -> output/1

== system acf_rl_native/Recenter travel ==
  note: Mid-stroke - actual travel
      | Deadband + slow gain + nominal robot path
      | Numerical step p.sim.step; sampling periods are independent.
  travel_m : Inport
  nominal_velocity : Inport  Port=2
  measured_force_error_N : Inport  Port=3
  Baseline or external robot : Switch  Criteria=u2 > Threshold  Threshold=.5  SaturateOnIntegerOverflow=off  InputSameDT=off
  Distance from mid stroke : Sum  Inputs=+-
  Force settling gate : Subsystem
  Gate contact or cell error : Switch  Criteria=u2 ~= 0  SaturateOnIntegerOverflow=off  InputSameDT=off
  Hold recentering : Constant  Value=0
  Measured or estimated travel : Switch  Criteria=u2 ~= 0  SaturateOnIntegerOverflow=off  InputSameDT=off
  Mid stroke : Constant  Value=p.mechanics.midTravel
  Nominal path sampling : ZeroOrderHold  SampleTime=p.robot.sampleTime
  RL fresh 100 Hz robot request : ZeroOrderHold  SampleTime=p.robot.sampleTime
  RL hard sign and gain envelope : sl_discontinuities/Saturation Dynamic  OutMin=[]  OutMax=[]  OutDataTypeStr=Inherit: Same as second input  OutDataType=fixdt(1, 16)  OutScaling=2^-10  DoSatur=off
      settings: LibrarySourceBlock=|
      | simulink/Discontinuities/Saturation
      | Dynamic
  RL negative recenter envelope : MinMax  Inputs=2
  RL positive recenter envelope : MinMax  Function=max  Inputs=2
  Recenter deadband : DeadZone  LowerValue=-p.robot.deadband  UpperValue=p.robot.deadband
  Recenter gain : Gain  Gain=p.uncertainty.recenterGain
  Robot feedback sampling : ZeroOrderHold  SampleTime=p.robot.sampleTime
  Robot speed limits : Saturate  UpperLimit=p.robot.maxSpeed  LowerLimit=-p.robot.maxSpeed
  Robot velocity request : Sum
  Send correction only when settled : Switch  Threshold=.5  SaturateOnIntegerOverflow=off  InputSameDT=off
  Tool sensor needs gap estimate : Constant  Value=p.sensor.positionModel
  Use reconstructed contact error : Constant  Value=double(p.sensor.distalMass_kg>0 && strcmp(p.actuator.kind,'voice_coil') && strcmp(p.coil.strategy,'observer'))
  requested_velocity : Outport
  tag scope: rl_baseline_robot=global, rl_force_gate=global, rl_issued_robot_correction=global, rl_issued_robot_total=global, rl_recenter_error=global
  wires:
  Mid stroke/1 -> Distance from mid stroke/1
  Robot feedback sampling/1 -> Distance from mid stroke/2
  nominal_velocity/1 -> Nominal path sampling/1
  Distance from mid stroke/1 -> Recenter deadband/1, [rl_recenter_error]
  Recenter deadband/1 -> Recenter gain/1
  Robot velocity request/1 -> Robot speed limits/1
  [nominal_velocity] -> Robot velocity request/1
  Nominal path sampling/1 -> [nominal_velocity]
  Recenter gain/1 -> [rl_baseline_robot], RL positive recenter envelope/1, RL negative recenter envelope/1, Baseline or external robot/1
  Force settling gate/1(ready) -> Send correction only when settled/2, [rl_force_gate]
  Hold recentering/1 -> Send correction only when settled/3, RL positive recenter envelope/2, RL negative recenter envelope/2
  Send correction only when settled/1 -> Robot velocity request/2, [rl_issued_robot_correction]
  Robot speed limits/1 -> requested_velocity/1, [rl_issued_robot_total]
  travel_m/1 -> Measured or estimated travel/3
  [estimated_actuator_travel_m] -> Measured or estimated travel/1
  Tool sensor needs gap estimate/1 -> Measured or estimated travel/2
  Measured or estimated travel/1 -> Robot feedback sampling/1
  measured_force_error_N/1 -> Gate contact or cell error/3
  [estimated_contact_error_N] -> Gate contact or cell error/1
  Use reconstructed contact error/1 -> Gate contact or cell error/2
  Gate contact or cell error/1 -> Force settling gate/1(force_error_N)
  [rl_external_robot] -> RL fresh 100 Hz robot request/1
  RL fresh 100 Hz robot request/1 -> RL hard sign and gain envelope/2
  RL positive recenter envelope/1 -> RL hard sign and gain envelope/1
  RL negative recenter envelope/1 -> RL hard sign and gain envelope/3
  [rl_baseline_mode] -> Baseline or external robot/2
  RL hard sign and gain envelope/1 -> Baseline or external robot/3
  Baseline or external robot/1 -> Send correction only when settled/1

== system acf_rl_native/Relative position measurement ==
  travel_m : Inport
  Coordinate reference : Constant  Value=p.mechanics.midTravel
  Measurement delay : Gain
  Position calibrated origin : Bias  Bias=p.d.positionMeasurementInitial  SaturateOnIntegerOverflow=off
  Position calibrated zero : Bias  Bias=-p.d.positionMeasurementInitial  SaturateOnIntegerOverflow=off
  Position noise : UniformRandomNumber  Minimum=-sqrt(3)  Maximum=sqrt(3)  Seed=p.sensor.seed+1  SampleTime=p.d.positionSampleTime
  Position noise RMS : Gain  Gain=p.adcStudy.d.positionNoiseInputRms_m
  Position sampling : ZeroOrderHold  SampleTime=p.d.positionSampleTime
  Residual position calibration : Gain  Gain=1+p.uncertainty.positionScale
  Select A and S : Selector  InputPortWidth=25  IndexOptions=Index vector (dialog)  Indices=[5 7]  OutputSizes=1
  Select position instrument : Switch  Criteria=u2 ~= 0  SaturateOnIntegerOverflow=off  InputSameDT=off
  Sensed position : Sum
  Tool S relative to A : Gain  Gain=[-1 1]  Multiplication=Matrix(K*u)
  Tool measurement coordinate : Sum
  Use toolhead position : Constant  Value=p.sensor.positionModel
  measured_travel_m : Outport
  wires:
  [plant_log] -> Select A and S/1
  Select A and S/1 -> Tool S relative to A/1
  Tool S relative to A/1 -> Tool measurement coordinate/1
  Coordinate reference/1 -> Tool measurement coordinate/2
  Tool measurement coordinate/1 -> Select position instrument/1
  Use toolhead position/1 -> Select position instrument/2
  travel_m/1 -> Select position instrument/3
  Position noise/1 -> Position noise RMS/1
  Position noise RMS/1 -> Sensed position/2
  Select position instrument/1 -> Position calibrated zero/1
  Position calibrated zero/1 -> Residual position calibration/1
  Residual position calibration/1 -> Position calibrated origin/1
  Position calibrated origin/1 -> Position sampling/1, Sensed position/1
  Sensed position/1 -> Measurement delay/1
  Measurement delay/1 -> measured_travel_m/1

== system acf_rl_native/Robot command delay ==
  note: Delay measured in robot command samples
      | Numerical step p.sim.step; sampling periods are independent.
  requested_velocity : Inport
  Held issued command at transport clock : ZeroOrderHold  SampleTime=p.d.actualRobotTransportSampleTime_s
  RL reset-fixed queue length : Constant  Value=p.d.robotDelaySamples
  Robot command samples : Delay  DelayLengthSource=Input port  DelayLength=p.d.robotDelaySamples  DelayLengthUpperLimit=1000  InitialCondition=p.robot.nominalVelocity*double(~p.robotPrediction.boundedNominalPath)  PreventDirectFeedthrough=on  DiagnosticForDelayLength=Error  UseCircularBuffer=on  SampleTime=p.d.actualRobotTransportSampleTime_s
      settings: InputPortMap=u0,p1
  delayed_velocity : Outport
  wires:
  Robot command samples/1 -> delayed_velocity/1
  requested_velocity/1 -> Held issued command at transport clock/1
  Held issued command at transport clock/1 -> Robot command samples/1
  RL reset-fixed queue length/1 -> Robot command samples/2

== system acf_rl_native/Robot motion ==
  note: Velocity response + speed/acceleration limits
      | Prescribed robot boundary, no robot force input
      | Numerical step p.sim.step; sampling periods are independent.
  delayed_velocity : Inport
  Requested robot speed : Saturate  UpperLimit=p.robot.maxSpeed  LowerLimit=-p.robot.maxSpeed
  Robot acceleration limits : Saturate  UpperLimit=p.robot.maxAcceleration  LowerLimit=-p.robot.maxAcceleration
  Robot position : Integrator  InitialCondition=p.d.r0
  Robot position and velocity : Mux  Inputs=2
  Robot speed error : Sum  Inputs=+-
  Robot velocity : Integrator
  Velocity response : Gain  Gain=1/p.robot.responseTime
  actual_r_v : Outport
  tag scope: robot_boundary_acceleration=global
  wires:
  delayed_velocity/1 -> Requested robot speed/1
  Velocity response/1 -> Robot acceleration limits/1
  Robot velocity/1 -> Robot position/1, [robot_velocity_m_s]
  [robot_position_m] -> Robot position and velocity/1
  [robot_velocity_m_s] -> Robot position and velocity/2
  Requested robot speed/1 -> Robot speed error/1
  [robot_velocity_m_s] -> Robot speed error/2
  Robot acceleration limits/1 -> Robot velocity/1, [robot_boundary_acceleration]
  Robot position/1 -> [robot_position_m]
  Robot speed error/1 -> Velocity response/1
  Robot position and velocity/1 -> actual_r_v/1
